simulink library "casper_library_correlator"  (Simulink 8.0)
settings: Solver=ode45  SolverMode=SingleTasking  StartTime=0.0  StopTime=10.0  RelTol=1e-3
values from neighbouring files (symbols this model uses):
  n_bits = eval(get_var('n_bits', 'defaults', defaults, varargin{:}))    [auto_tap_init.m]    (also in baseline_tap_init.m; bi_real_unscr_2x_init.m = get_var('n_bits', 'defaults', defaults, varargin{:}); bi_real_unscr_4x_init.m = get_var('n_bits', 'defaults', defaults, varargin{:}); bit_reverse_init.m = get_var('n_bits',varargin{:}))
libraries: xbsIndex_r4 x1360, casper_library_misc x140, casper_library_multipliers x32, xps_library x8, casper_library_delays x1, casper_library_correlator x1
(part 2 of 14)

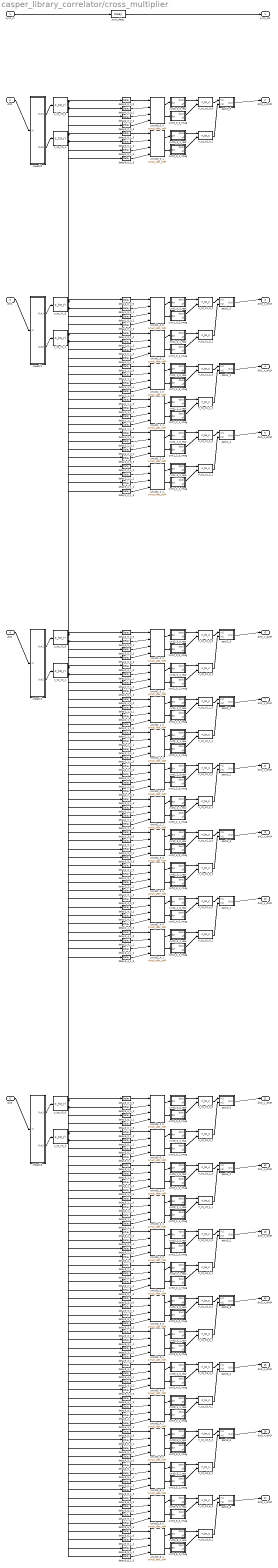
== system casper_library_correlator/cross_multiplier ==
  sync_in : Inport
  din0 : Inport  Port=2
  din1 : Inport  Port=3
  din2 : Inport  Port=4
  din3 : Inport  Port=5
  c_to_ri0_0 : casper_library_misc/c_to_ri  n_bits=bit_width_in  bin_pt=binary_point_in
      settings: AttributesFormatString=4_3 r/i
  c_to_ri0_1 : casper_library_misc/c_to_ri  n_bits=bit_width_in  bin_pt=binary_point_in
      settings: AttributesFormatString=4_3 r/i
  c_to_ri1_0 : casper_library_misc/c_to_ri  n_bits=bit_width_in  bin_pt=binary_point_in
      settings: AttributesFormatString=4_3 r/i
  c_to_ri1_1 : casper_library_misc/c_to_ri  n_bits=bit_width_in  bin_pt=binary_point_in
      settings: AttributesFormatString=4_3 r/i
  c_to_ri2_0 : casper_library_misc/c_to_ri  n_bits=bit_width_in  bin_pt=binary_point_in
      settings: AttributesFormatString=4_3 r/i
  c_to_ri2_1 : casper_library_misc/c_to_ri  n_bits=bit_width_in  bin_pt=binary_point_in
      settings: AttributesFormatString=4_3 r/i
  c_to_ri3_0 : casper_library_misc/c_to_ri  n_bits=bit_width_in  bin_pt=binary_point_in
      settings: AttributesFormatString=4_3 r/i
  c_to_ri3_1 : casper_library_misc/c_to_ri  n_bits=bit_width_in  bin_pt=binary_point_in
      settings: AttributesFormatString=4_3 r/i
  cmult0_0_0 : casper_library_multipliers/cmult_4bit_hdl*  mult_latency=mult_latency  add_latency=add_latency
  cmult0_0_1 : casper_library_multipliers/cmult_4bit_hdl*  mult_latency=mult_latency  add_latency=add_latency
  cmult1_0_0 : casper_library_multipliers/cmult_4bit_hdl*  mult_latency=mult_latency  add_latency=add_latency
  cmult1_0_1 : casper_library_multipliers/cmult_4bit_hdl*  mult_latency=mult_latency  add_latency=add_latency
  cmult1_1_0 : casper_library_multipliers/cmult_4bit_hdl*  mult_latency=mult_latency  add_latency=add_latency
  cmult1_1_1 : casper_library_multipliers/cmult_4bit_hdl*  mult_latency=mult_latency  add_latency=add_latency
  cmult1_2_0 : casper_library_multipliers/cmult_4bit_hdl*  mult_latency=mult_latency  add_latency=add_latency
  cmult1_2_1 : casper_library_multipliers/cmult_4bit_hdl*  mult_latency=mult_latency  add_latency=add_latency
  cmult2_0_0 : casper_library_multipliers/cmult_4bit_hdl*  mult_latency=mult_latency  add_latency=add_latency
  cmult2_0_1 : casper_library_multipliers/cmult_4bit_hdl*  mult_latency=mult_latency  add_latency=add_latency
  cmult2_1_0 : casper_library_multipliers/cmult_4bit_hdl*  mult_latency=mult_latency  add_latency=add_latency
  cmult2_1_1 : casper_library_multipliers/cmult_4bit_hdl*  mult_latency=mult_latency  add_latency=add_latency
  cmult2_2_0 : casper_library_multipliers/cmult_4bit_hdl*  mult_latency=mult_latency  add_latency=add_latency
  cmult2_2_1 : casper_library_multipliers/cmult_4bit_hdl*  mult_latency=mult_latency  add_latency=add_latency
  cmult2_3_0 : casper_library_multipliers/cmult_4bit_hdl*  mult_latency=mult_latency  add_latency=add_latency
  cmult2_3_1 : casper_library_multipliers/cmult_4bit_hdl*  mult_latency=mult_latency  add_latency=add_latency
  cmult2_4_0 : casper_library_multipliers/cmult_4bit_hdl*  mult_latency=mult_latency  add_latency=add_latency
  cmult2_4_1 : casper_library_multipliers/cmult_4bit_hdl*  mult_latency=mult_latency  add_latency=add_latency
  cmult3_0_0 : casper_library_multipliers/cmult_4bit_hdl*  mult_latency=mult_latency  add_latency=add_latency
  cmult3_0_1 : casper_library_multipliers/cmult_4bit_hdl*  mult_latency=mult_latency  add_latency=add_latency
  cmult3_1_0 : casper_library_multipliers/cmult_4bit_hdl*  mult_latency=mult_latency  add_latency=add_latency
  cmult3_1_1 : casper_library_multipliers/cmult_4bit_hdl*  mult_latency=mult_latency  add_latency=add_latency
  cmult3_2_0 : casper_library_multipliers/cmult_4bit_hdl*  mult_latency=mult_latency  add_latency=add_latency
  cmult3_2_1 : casper_library_multipliers/cmult_4bit_hdl*  mult_latency=mult_latency  add_latency=add_latency
  cmult3_3_0 : casper_library_multipliers/cmult_4bit_hdl*  mult_latency=mult_latency  add_latency=add_latency
  cmult3_3_1 : casper_library_multipliers/cmult_4bit_hdl*  mult_latency=mult_latency  add_latency=add_latency
  cmult3_4_0 : casper_library_multipliers/cmult_4bit_hdl*  mult_latency=mult_latency  add_latency=add_latency
  cmult3_4_1 : casper_library_multipliers/cmult_4bit_hdl*  mult_latency=mult_latency  add_latency=add_latency
  cmult3_5_0 : casper_library_multipliers/cmult_4bit_hdl*  mult_latency=mult_latency  add_latency=add_latency
  cmult3_5_1 : casper_library_multipliers/cmult_4bit_hdl*  mult_latency=mult_latency  add_latency=add_latency
  cmult3_6_0 : casper_library_multipliers/cmult_4bit_hdl*  mult_latency=mult_latency  add_latency=add_latency
  cmult3_6_1 : casper_library_multipliers/cmult_4bit_hdl*  mult_latency=mult_latency  add_latency=add_latency
  cvrt0_0_0_imag : Subsystem  AncestorBlock=casper_library_misc/convert_of  mask(convert_of){bit_width_i=9, binary_point_i=6, bit_width_o=9, binary_point_o=6, latency=0, overflow=Wrap, quantization=Truncate}
      mask prompts: bit_width_i "Bit Width In"; binary_point_i "Binary Point In"; bit_width_o "Bit Width Out"; binary_point_o "Binary Point Out"; overflow "Overflow Behaviour"; quantization "Quantization Behaviour"
      mask help:
      | Converts from one 2's complement bit-width
      | and/or binary point position to another.
      | Includes underflow/overflow indicator.
      mask init:
      | convert_of_init(gcb, ...
      |     'bit_width_i', bit_width_i, ...
      |     'binary_point_i', binary_point_i, ...
      |     'bit_width_o', bit_width_o, ...
      |     'binary_point_o', binary_point_o, ...
      |     'latency', latency, ...
      |     'overflow', overflow, ...
      |     'quantization', quantization);
      settings: AttributesFormatString=[9,6]->[9,6]
      mask TypeOptions overflow: Wrap | Saturate | Error
      mask TypeOptions quantization: Truncate | Round  (unbiased: +/- Inf) | Round  (unbiased: even values)
  cvrt0_0_0_real : Subsystem  AncestorBlock=casper_library_misc/convert_of  mask(convert_of){bit_width_i=9, binary_point_i=6, bit_width_o=9, binary_point_o=6, latency=0, overflow=Wrap, quantization=Truncate}
      mask prompts: bit_width_i "Bit Width In"; binary_point_i "Binary Point In"; bit_width_o "Bit Width Out"; binary_point_o "Binary Point Out"; overflow "Overflow Behaviour"; quantization "Quantization Behaviour"
      mask help:
      | Converts from one 2's complement bit-width
      | and/or binary point position to another.
      | Includes underflow/overflow indicator.
      mask init: same as casper_library_correlator/cross_multiplier/cvrt0_0_0_imag
      settings: AttributesFormatString=[9,6]->[9,6]
      mask TypeOptions overflow: Wrap | Saturate | Error
      mask TypeOptions quantization: Truncate | Round  (unbiased: +/- Inf) | Round  (unbiased: even values)
  cvrt0_0_1_imag : Subsystem  AncestorBlock=casper_library_misc/convert_of  mask(convert_of){bit_width_i=9, binary_point_i=6, bit_width_o=9, binary_point_o=6, latency=0, overflow=Wrap, quantization=Truncate}
      mask prompts: bit_width_i "Bit Width In"; binary_point_i "Binary Point In"; bit_width_o "Bit Width Out"; binary_point_o "Binary Point Out"; overflow "Overflow Behaviour"; quantization "Quantization Behaviour"
      mask help:
      | Converts from one 2's complement bit-width
      | and/or binary point position to another.
      | Includes underflow/overflow indicator.
      mask init: same as casper_library_correlator/cross_multiplier/cvrt0_0_0_imag
      settings: AttributesFormatString=[9,6]->[9,6]
      mask TypeOptions overflow: Wrap | Saturate | Error
      mask TypeOptions quantization: Truncate | Round  (unbiased: +/- Inf) | Round  (unbiased: even values)
  cvrt0_0_1_real : Subsystem  AncestorBlock=casper_library_misc/convert_of  mask(convert_of){bit_width_i=9, binary_point_i=6, bit_width_o=9, binary_point_o=6, latency=0, overflow=Wrap, quantization=Truncate}
      mask prompts: bit_width_i "Bit Width In"; binary_point_i "Binary Point In"; bit_width_o "Bit Width Out"; binary_point_o "Binary Point Out"; overflow "Overflow Behaviour"; quantization "Quantization Behaviour"
      mask help:
      | Converts from one 2's complement bit-width
      | and/or binary point position to another.
      | Includes underflow/overflow indicator.
      mask init: same as casper_library_correlator/cross_multiplier/cvrt0_0_0_imag
      settings: AttributesFormatString=[9,6]->[9,6]
      mask TypeOptions overflow: Wrap | Saturate | Error
      mask TypeOptions quantization: Truncate | Round  (unbiased: +/- Inf) | Round  (unbiased: even values)
  cvrt1_0_0_imag : Subsystem  AncestorBlock=casper_library_misc/convert_of  mask(convert_of){bit_width_i=9, binary_point_i=6, bit_width_o=9, binary_point_o=6, latency=0, overflow=Wrap, quantization=Truncate}
      mask prompts: bit_width_i "Bit Width In"; binary_point_i "Binary Point In"; bit_width_o "Bit Width Out"; binary_point_o "Binary Point Out"; overflow "Overflow Behaviour"; quantization "Quantization Behaviour"
      mask help:
      | Converts from one 2's complement bit-width
      | and/or binary point position to another.
      | Includes underflow/overflow indicator.
      mask init: same as casper_library_correlator/cross_multiplier/cvrt0_0_0_imag
      settings: AttributesFormatString=[9,6]->[9,6]
      mask TypeOptions overflow: Wrap | Saturate | Error
      mask TypeOptions quantization: Truncate | Round  (unbiased: +/- Inf) | Round  (unbiased: even values)
  cvrt1_0_0_real : Subsystem  AncestorBlock=casper_library_misc/convert_of  mask(convert_of){bit_width_i=9, binary_point_i=6, bit_width_o=9, binary_point_o=6, latency=0, overflow=Wrap, quantization=Truncate}
      mask prompts: bit_width_i "Bit Width In"; binary_point_i "Binary Point In"; bit_width_o "Bit Width Out"; binary_point_o "Binary Point Out"; overflow "Overflow Behaviour"; quantization "Quantization Behaviour"
      mask help:
      | Converts from one 2's complement bit-width
      | and/or binary point position to another.
      | Includes underflow/overflow indicator.
      mask init: same as casper_library_correlator/cross_multiplier/cvrt0_0_0_imag
      settings: AttributesFormatString=[9,6]->[9,6]
      mask TypeOptions overflow: Wrap | Saturate | Error
      mask TypeOptions quantization: Truncate | Round  (unbiased: +/- Inf) | Round  (unbiased: even values)
  cvrt1_0_1_imag : Subsystem  AncestorBlock=casper_library_misc/convert_of  mask(convert_of){bit_width_i=9, binary_point_i=6, bit_width_o=9, binary_point_o=6, latency=0, overflow=Wrap, quantization=Truncate}
      mask prompts: bit_width_i "Bit Width In"; binary_point_i "Binary Point In"; bit_width_o "Bit Width Out"; binary_point_o "Binary Point Out"; overflow "Overflow Behaviour"; quantization "Quantization Behaviour"
      mask help:
      | Converts from one 2's complement bit-width
      | and/or binary point position to another.
      | Includes underflow/overflow indicator.
      mask init: same as casper_library_correlator/cross_multiplier/cvrt0_0_0_imag
      settings: AttributesFormatString=[9,6]->[9,6]
      mask TypeOptions overflow: Wrap | Saturate | Error
      mask TypeOptions quantization: Truncate | Round  (unbiased: +/- Inf) | Round  (unbiased: even values)
  cvrt1_0_1_real : Subsystem  AncestorBlock=casper_library_misc/convert_of  mask(convert_of){bit_width_i=9, binary_point_i=6, bit_width_o=9, binary_point_o=6, latency=0, overflow=Wrap, quantization=Truncate}
      mask prompts: bit_width_i "Bit Width In"; binary_point_i "Binary Point In"; bit_width_o "Bit Width Out"; binary_point_o "Binary Point Out"; overflow "Overflow Behaviour"; quantization "Quantization Behaviour"
      mask help:
      | Converts from one 2's complement bit-width
      | and/or binary point position to another.
      | Includes underflow/overflow indicator.
      mask init: same as casper_library_correlator/cross_multiplier/cvrt0_0_0_imag
      settings: AttributesFormatString=[9,6]->[9,6]
      mask TypeOptions overflow: Wrap | Saturate | Error
      mask TypeOptions quantization: Truncate | Round  (unbiased: +/- Inf) | Round  (unbiased: even values)
  cvrt1_1_0_imag : Subsystem  AncestorBlock=casper_library_misc/convert_of  mask(convert_of){bit_width_i=9, binary_point_i=6, bit_width_o=9, binary_point_o=6, latency=0, overflow=Wrap, quantization=Truncate}
      mask prompts: bit_width_i "Bit Width In"; binary_point_i "Binary Point In"; bit_width_o "Bit Width Out"; binary_point_o "Binary Point Out"; overflow "Overflow Behaviour"; quantization "Quantization Behaviour"
      mask help:
      | Converts from one 2's complement bit-width
      | and/or binary point position to another.
      | Includes underflow/overflow indicator.
      mask init: same as casper_library_correlator/cross_multiplier/cvrt0_0_0_imag
      settings: AttributesFormatString=[9,6]->[9,6]
      mask TypeOptions overflow: Wrap | Saturate | Error
      mask TypeOptions quantization: Truncate | Round  (unbiased: +/- Inf) | Round  (unbiased: even values)
  cvrt1_1_0_real : Subsystem  AncestorBlock=casper_library_misc/convert_of  mask(convert_of){bit_width_i=9, binary_point_i=6, bit_width_o=9, binary_point_o=6, latency=0, overflow=Wrap, quantization=Truncate}
      mask prompts: bit_width_i "Bit Width In"; binary_point_i "Binary Point In"; bit_width_o "Bit Width Out"; binary_point_o "Binary Point Out"; overflow "Overflow Behaviour"; quantization "Quantization Behaviour"
      mask help:
      | Converts from one 2's complement bit-width
      | and/or binary point position to another.
      | Includes underflow/overflow indicator.
      mask init: same as casper_library_correlator/cross_multiplier/cvrt0_0_0_imag
      settings: AttributesFormatString=[9,6]->[9,6]
      mask TypeOptions overflow: Wrap | Saturate | Error
      mask TypeOptions quantization: Truncate | Round  (unbiased: +/- Inf) | Round  (unbiased: even values)
  cvrt1_1_1_imag : Subsystem  AncestorBlock=casper_library_misc/convert_of  mask(convert_of){bit_width_i=9, binary_point_i=6, bit_width_o=9, binary_point_o=6, latency=0, overflow=Wrap, quantization=Truncate}
      mask prompts: bit_width_i "Bit Width In"; binary_point_i "Binary Point In"; bit_width_o "Bit Width Out"; binary_point_o "Binary Point Out"; overflow "Overflow Behaviour"; quantization "Quantization Behaviour"
      mask help:
      | Converts from one 2's complement bit-width
      | and/or binary point position to another.
      | Includes underflow/overflow indicator.
      mask init: same as casper_library_correlator/cross_multiplier/cvrt0_0_0_imag
      settings: AttributesFormatString=[9,6]->[9,6]
      mask TypeOptions overflow: Wrap | Saturate | Error
      mask TypeOptions quantization: Truncate | Round  (unbiased: +/- Inf) | Round  (unbiased: even values)
  cvrt1_1_1_real : Subsystem  AncestorBlock=casper_library_misc/convert_of  mask(convert_of){bit_width_i=9, binary_point_i=6, bit_width_o=9, binary_point_o=6, latency=0, overflow=Wrap, quantization=Truncate}
      mask prompts: bit_width_i "Bit Width In"; binary_point_i "Binary Point In"; bit_width_o "Bit Width Out"; binary_point_o "Binary Point Out"; overflow "Overflow Behaviour"; quantization "Quantization Behaviour"
      mask help:
      | Converts from one 2's complement bit-width
      | and/or binary point position to another.
      | Includes underflow/overflow indicator.
      mask init: same as casper_library_correlator/cross_multiplier/cvrt0_0_0_imag
      settings: AttributesFormatString=[9,6]->[9,6]
      mask TypeOptions overflow: Wrap | Saturate | Error
      mask TypeOptions quantization: Truncate | Round  (unbiased: +/- Inf) | Round  (unbiased: even values)
  cvrt1_2_0_imag : Subsystem  AncestorBlock=casper_library_misc/convert_of  mask(convert_of){bit_width_i=9, binary_point_i=6, bit_width_o=9, binary_point_o=6, latency=0, overflow=Wrap, quantization=Truncate}
      mask prompts: bit_width_i "Bit Width In"; binary_point_i "Binary Point In"; bit_width_o "Bit Width Out"; binary_point_o "Binary Point Out"; overflow "Overflow Behaviour"; quantization "Quantization Behaviour"
      mask help:
      | Converts from one 2's complement bit-width
      | and/or binary point position to another.
      | Includes underflow/overflow indicator.
      mask init: same as casper_library_correlator/cross_multiplier/cvrt0_0_0_imag
      settings: AttributesFormatString=[9,6]->[9,6]
      mask TypeOptions overflow: Wrap | Saturate | Error
      mask TypeOptions quantization: Truncate | Round  (unbiased: +/- Inf) | Round  (unbiased: even values)
  cvrt1_2_0_real : Subsystem  AncestorBlock=casper_library_misc/convert_of  mask(convert_of){bit_width_i=9, binary_point_i=6, bit_width_o=9, binary_point_o=6, latency=0, overflow=Wrap, quantization=Truncate}
      mask prompts: bit_width_i "Bit Width In"; binary_point_i "Binary Point In"; bit_width_o "Bit Width Out"; binary_point_o "Binary Point Out"; overflow "Overflow Behaviour"; quantization "Quantization Behaviour"
      mask help:
      | Converts from one 2's complement bit-width
      | and/or binary point position to another.
      | Includes underflow/overflow indicator.
      mask init: same as casper_library_correlator/cross_multiplier/cvrt0_0_0_imag
      settings: AttributesFormatString=[9,6]->[9,6]
      mask TypeOptions overflow: Wrap | Saturate | Error
      mask TypeOptions quantization: Truncate | Round  (unbiased: +/- Inf) | Round  (unbiased: even values)
  cvrt1_2_1_imag : Subsystem  AncestorBlock=casper_library_misc/convert_of  mask(convert_of){bit_width_i=9, binary_point_i=6, bit_width_o=9, binary_point_o=6, latency=0, overflow=Wrap, quantization=Truncate}
      mask prompts: bit_width_i "Bit Width In"; binary_point_i "Binary Point In"; bit_width_o "Bit Width Out"; binary_point_o "Binary Point Out"; overflow "Overflow Behaviour"; quantization "Quantization Behaviour"
      mask help:
      | Converts from one 2's complement bit-width
      | and/or binary point position to another.
      | Includes underflow/overflow indicator.
      mask init: same as casper_library_correlator/cross_multiplier/cvrt0_0_0_imag
      settings: AttributesFormatString=[9,6]->[9,6]
      mask TypeOptions overflow: Wrap | Saturate | Error
      mask TypeOptions quantization: Truncate | Round  (unbiased: +/- Inf) | Round  (unbiased: even values)
  cvrt1_2_1_real : Subsystem  AncestorBlock=casper_library_misc/convert_of  mask(convert_of){bit_width_i=9, binary_point_i=6, bit_width_o=9, binary_point_o=6, latency=0, overflow=Wrap, quantization=Truncate}
      mask prompts: bit_width_i "Bit Width In"; binary_point_i "Binary Point In"; bit_width_o "Bit Width Out"; binary_point_o "Binary Point Out"; overflow "Overflow Behaviour"; quantization "Quantization Behaviour"
      mask help:
      | Converts from one 2's complement bit-width
      | and/or binary point position to another.
      | Includes underflow/overflow indicator.
      mask init: same as casper_library_correlator/cross_multiplier/cvrt0_0_0_imag
      settings: AttributesFormatString=[9,6]->[9,6]
      mask TypeOptions overflow: Wrap | Saturate | Error
      mask TypeOptions quantization: Truncate | Round  (unbiased: +/- Inf) | Round  (unbiased: even values)
  cvrt2_0_0_imag : Subsystem  AncestorBlock=casper_library_misc/convert_of  mask(convert_of){bit_width_i=9, binary_point_i=6, bit_width_o=9, binary_point_o=6, latency=0, overflow=Wrap, quantization=Truncate}
      mask prompts: bit_width_i "Bit Width In"; binary_point_i "Binary Point In"; bit_width_o "Bit Width Out"; binary_point_o "Binary Point Out"; overflow "Overflow Behaviour"; quantization "Quantization Behaviour"
      mask help:
      | Converts from one 2's complement bit-width
      | and/or binary point position to another.
      | Includes underflow/overflow indicator.
      mask init: same as casper_library_correlator/cross_multiplier/cvrt0_0_0_imag
      settings: AttributesFormatString=[9,6]->[9,6]
      mask TypeOptions overflow: Wrap | Saturate | Error
      mask TypeOptions quantization: Truncate | Round  (unbiased: +/- Inf) | Round  (unbiased: even values)
  cvrt2_0_0_real : Subsystem  AncestorBlock=casper_library_misc/convert_of  mask(convert_of){bit_width_i=9, binary_point_i=6, bit_width_o=9, binary_point_o=6, latency=0, overflow=Wrap, quantization=Truncate}
      mask prompts: bit_width_i "Bit Width In"; binary_point_i "Binary Point In"; bit_width_o "Bit Width Out"; binary_point_o "Binary Point Out"; overflow "Overflow Behaviour"; quantization "Quantization Behaviour"
      mask help:
      | Converts from one 2's complement bit-width
      | and/or binary point position to another.
      | Includes underflow/overflow indicator.
      mask init: same as casper_library_correlator/cross_multiplier/cvrt0_0_0_imag
      settings: AttributesFormatString=[9,6]->[9,6]
      mask TypeOptions overflow: Wrap | Saturate | Error
      mask TypeOptions quantization: Truncate | Round  (unbiased: +/- Inf) | Round  (unbiased: even values)
  cvrt2_0_1_imag : Subsystem  AncestorBlock=casper_library_misc/convert_of  mask(convert_of){bit_width_i=9, binary_point_i=6, bit_width_o=9, binary_point_o=6, latency=0, overflow=Wrap, quantization=Truncate}
      mask prompts: bit_width_i "Bit Width In"; binary_point_i "Binary Point In"; bit_width_o "Bit Width Out"; binary_point_o "Binary Point Out"; overflow "Overflow Behaviour"; quantization "Quantization Behaviour"
      mask help:
      | Converts from one 2's complement bit-width
      | and/or binary point position to another.
      | Includes underflow/overflow indicator.
      mask init: same as casper_library_correlator/cross_multiplier/cvrt0_0_0_imag
      settings: AttributesFormatString=[9,6]->[9,6]
      mask TypeOptions overflow: Wrap | Saturate | Error
      mask TypeOptions quantization: Truncate | Round  (unbiased: +/- Inf) | Round  (unbiased: even values)
  cvrt2_0_1_real : Subsystem  AncestorBlock=casper_library_misc/convert_of  mask(convert_of){bit_width_i=9, binary_point_i=6, bit_width_o=9, binary_point_o=6, latency=0, overflow=Wrap, quantization=Truncate}
      mask prompts: bit_width_i "Bit Width In"; binary_point_i "Binary Point In"; bit_width_o "Bit Width Out"; binary_point_o "Binary Point Out"; overflow "Overflow Behaviour"; quantization "Quantization Behaviour"
      mask help:
      | Converts from one 2's complement bit-width
      | and/or binary point position to another.
      | Includes underflow/overflow indicator.
      mask init: same as casper_library_correlator/cross_multiplier/cvrt0_0_0_imag
      settings: AttributesFormatString=[9,6]->[9,6]
      mask TypeOptions overflow: Wrap | Saturate | Error
      mask TypeOptions quantization: Truncate | Round  (unbiased: +/- Inf) | Round  (unbiased: even values)
  cvrt2_1_0_imag : Subsystem  AncestorBlock=casper_library_misc/convert_of  mask(convert_of){bit_width_i=9, binary_point_i=6, bit_width_o=9, binary_point_o=6, latency=0, overflow=Wrap, quantization=Truncate}
      mask prompts: bit_width_i "Bit Width In"; binary_point_i "Binary Point In"; bit_width_o "Bit Width Out"; binary_point_o "Binary Point Out"; overflow "Overflow Behaviour"; quantization "Quantization Behaviour"
      mask help:
      | Converts from one 2's complement bit-width
      | and/or binary point position to another.
      | Includes underflow/overflow indicator.
      mask init: same as casper_library_correlator/cross_multiplier/cvrt0_0_0_imag
      settings: AttributesFormatString=[9,6]->[9,6]
      mask TypeOptions overflow: Wrap | Saturate | Error
      mask TypeOptions quantization: Truncate | Round  (unbiased: +/- Inf) | Round  (unbiased: even values)
  cvrt2_1_0_real : Subsystem  AncestorBlock=casper_library_misc/convert_of  mask(convert_of){bit_width_i=9, binary_point_i=6, bit_width_o=9, binary_point_o=6, latency=0, overflow=Wrap, quantization=Truncate}
      mask prompts: bit_width_i "Bit Width In"; binary_point_i "Binary Point In"; bit_width_o "Bit Width Out"; binary_point_o "Binary Point Out"; overflow "Overflow Behaviour"; quantization "Quantization Behaviour"
      mask help:
      | Converts from one 2's complement bit-width
      | and/or binary point position to another.
      | Includes underflow/overflow indicator.
      mask init: same as casper_library_correlator/cross_multiplier/cvrt0_0_0_imag
      settings: AttributesFormatString=[9,6]->[9,6]
      mask TypeOptions overflow: Wrap | Saturate | Error
      mask TypeOptions quantization: Truncate | Round  (unbiased: +/- Inf) | Round  (unbiased: even values)
  cvrt2_1_1_imag : Subsystem  AncestorBlock=casper_library_misc/convert_of  mask(convert_of){bit_width_i=9, binary_point_i=6, bit_width_o=9, binary_point_o=6, latency=0, overflow=Wrap, quantization=Truncate}
      mask prompts: bit_width_i "Bit Width In"; binary_point_i "Binary Point In"; bit_width_o "Bit Width Out"; binary_point_o "Binary Point Out"; overflow "Overflow Behaviour"; quantization "Quantization Behaviour"
      mask help:
      | Converts from one 2's complement bit-width
      | and/or binary point position to another.
      | Includes underflow/overflow indicator.
      mask init: same as casper_library_correlator/cross_multiplier/cvrt0_0_0_imag
      settings: AttributesFormatString=[9,6]->[9,6]
      mask TypeOptions overflow: Wrap | Saturate | Error
      mask TypeOptions quantization: Truncate | Round  (unbiased: +/- Inf) | Round  (unbiased: even values)
  cvrt2_1_1_real : Subsystem  AncestorBlock=casper_library_misc/convert_of  mask(convert_of){bit_width_i=9, binary_point_i=6, bit_width_o=9, binary_point_o=6, latency=0, overflow=Wrap, quantization=Truncate}
      mask prompts: bit_width_i "Bit Width In"; binary_point_i "Binary Point In"; bit_width_o "Bit Width Out"; binary_point_o "Binary Point Out"; overflow "Overflow Behaviour"; quantization "Quantization Behaviour"
      mask help:
      | Converts from one 2's complement bit-width
      | and/or binary point position to another.
      | Includes underflow/overflow indicator.
      mask init: same as casper_library_correlator/cross_multiplier/cvrt0_0_0_imag
      settings: AttributesFormatString=[9,6]->[9,6]
      mask TypeOptions overflow: Wrap | Saturate | Error
      mask TypeOptions quantization: Truncate | Round  (unbiased: +/- Inf) | Round  (unbiased: even values)
  cvrt2_2_0_imag : Subsystem  AncestorBlock=casper_library_misc/convert_of  mask(convert_of){bit_width_i=9, binary_point_i=6, bit_width_o=9, binary_point_o=6, latency=0, overflow=Wrap, quantization=Truncate}
      mask prompts: bit_width_i "Bit Width In"; binary_point_i "Binary Point In"; bit_width_o "Bit Width Out"; binary_point_o "Binary Point Out"; overflow "Overflow Behaviour"; quantization "Quantization Behaviour"
      mask help:
      | Converts from one 2's complement bit-width
      | and/or binary point position to another.
      | Includes underflow/overflow indicator.
      mask init: same as casper_library_correlator/cross_multiplier/cvrt0_0_0_imag
      settings: AttributesFormatString=[9,6]->[9,6]
      mask TypeOptions overflow: Wrap | Saturate | Error
      mask TypeOptions quantization: Truncate | Round  (unbiased: +/- Inf) | Round  (unbiased: even values)
  cvrt2_2_0_real : Subsystem  AncestorBlock=casper_library_misc/convert_of  mask(convert_of){bit_width_i=9, binary_point_i=6, bit_width_o=9, binary_point_o=6, latency=0, overflow=Wrap, quantization=Truncate}
      mask prompts: bit_width_i "Bit Width In"; binary_point_i "Binary Point In"; bit_width_o "Bit Width Out"; binary_point_o "Binary Point Out"; overflow "Overflow Behaviour"; quantization "Quantization Behaviour"
      mask help:
      | Converts from one 2's complement bit-width
      | and/or binary point position to another.
      | Includes underflow/overflow indicator.
      mask init: same as casper_library_correlator/cross_multiplier/cvrt0_0_0_imag
      settings: AttributesFormatString=[9,6]->[9,6]
      mask TypeOptions overflow: Wrap | Saturate | Error
      mask TypeOptions quantization: Truncate | Round  (unbiased: +/- Inf) | Round  (unbiased: even values)
  cvrt2_2_1_imag : Subsystem  AncestorBlock=casper_library_misc/convert_of  mask(convert_of){bit_width_i=9, binary_point_i=6, bit_width_o=9, binary_point_o=6, latency=0, overflow=Wrap, quantization=Truncate}
      mask prompts: bit_width_i "Bit Width In"; binary_point_i "Binary Point In"; bit_width_o "Bit Width Out"; binary_point_o "Binary Point Out"; overflow "Overflow Behaviour"; quantization "Quantization Behaviour"
      mask help:
      | Converts from one 2's complement bit-width
      | and/or binary point position to another.
      | Includes underflow/overflow indicator.
      mask init: same as casper_library_correlator/cross_multiplier/cvrt0_0_0_imag
      settings: AttributesFormatString=[9,6]->[9,6]
      mask TypeOptions overflow: Wrap | Saturate | Error
      mask TypeOptions quantization: Truncate | Round  (unbiased: +/- Inf) | Round  (unbiased: even values)
  cvrt2_2_1_real : Subsystem  AncestorBlock=casper_library_misc/convert_of  mask(convert_of){bit_width_i=9, binary_point_i=6, bit_width_o=9, binary_point_o=6, latency=0, overflow=Wrap, quantization=Truncate}
      mask prompts: bit_width_i "Bit Width In"; binary_point_i "Binary Point In"; bit_width_o "Bit Width Out"; binary_point_o "Binary Point Out"; overflow "Overflow Behaviour"; quantization "Quantization Behaviour"
      mask help:
      | Converts from one 2's complement bit-width
      | and/or binary point position to another.
      | Includes underflow/overflow indicator.
      mask init: same as casper_library_correlator/cross_multiplier/cvrt0_0_0_imag
      settings: AttributesFormatString=[9,6]->[9,6]
      mask TypeOptions overflow: Wrap | Saturate | Error
      mask TypeOptions quantization: Truncate | Round  (unbiased: +/- Inf) | Round  (unbiased: even values)
  cvrt2_3_0_imag : Subsystem  AncestorBlock=casper_library_misc/convert_of  mask(convert_of){bit_width_i=9, binary_point_i=6, bit_width_o=9, binary_point_o=6, latency=0, overflow=Wrap, quantization=Truncate}
      mask prompts: bit_width_i "Bit Width In"; binary_point_i "Binary Point In"; bit_width_o "Bit Width Out"; binary_point_o "Binary Point Out"; overflow "Overflow Behaviour"; quantization "Quantization Behaviour"
      mask help:
      | Converts from one 2's complement bit-width
      | and/or binary point position to another.
      | Includes underflow/overflow indicator.
      mask init: same as casper_library_correlator/cross_multiplier/cvrt0_0_0_imag
      settings: AttributesFormatString=[9,6]->[9,6]
      mask TypeOptions overflow: Wrap | Saturate | Error
      mask TypeOptions quantization: Truncate | Round  (unbiased: +/- Inf) | Round  (unbiased: even values)
  cvrt2_3_0_real : Subsystem  AncestorBlock=casper_library_misc/convert_of  mask(convert_of){bit_width_i=9, binary_point_i=6, bit_width_o=9, binary_point_o=6, latency=0, overflow=Wrap, quantization=Truncate}
      mask prompts: bit_width_i "Bit Width In"; binary_point_i "Binary Point In"; bit_width_o "Bit Width Out"; binary_point_o "Binary Point Out"; overflow "Overflow Behaviour"; quantization "Quantization Behaviour"
      mask help:
      | Converts from one 2's complement bit-width
      | and/or binary point position to another.
      | Includes underflow/overflow indicator.
      mask init: same as casper_library_correlator/cross_multiplier/cvrt0_0_0_imag
      settings: AttributesFormatString=[9,6]->[9,6]
      mask TypeOptions overflow: Wrap | Saturate | Error
      mask TypeOptions quantization: Truncate | Round  (unbiased: +/- Inf) | Round  (unbiased: even values)
  cvrt2_3_1_imag : Subsystem  AncestorBlock=casper_library_misc/convert_of  mask(convert_of){bit_width_i=9, binary_point_i=6, bit_width_o=9, binary_point_o=6, latency=0, overflow=Wrap, quantization=Truncate}
      mask prompts: bit_width_i "Bit Width In"; binary_point_i "Binary Point In"; bit_width_o "Bit Width Out"; binary_point_o "Binary Point Out"; overflow "Overflow Behaviour"; quantization "Quantization Behaviour"
      mask help:
      | Converts from one 2's complement bit-width
      | and/or binary point position to another.
      | Includes underflow/overflow indicator.
      mask init: same as casper_library_correlator/cross_multiplier/cvrt0_0_0_imag
      settings: AttributesFormatString=[9,6]->[9,6]
      mask TypeOptions overflow: Wrap | Saturate | Error
      mask TypeOptions quantization: Truncate | Round  (unbiased: +/- Inf) | Round  (unbiased: even values)
  cvrt2_3_1_real : Subsystem  AncestorBlock=casper_library_misc/convert_of  mask(convert_of){bit_width_i=9, binary_point_i=6, bit_width_o=9, binary_point_o=6, latency=0, overflow=Wrap, quantization=Truncate}
      mask prompts: bit_width_i "Bit Width In"; binary_point_i "Binary Point In"; bit_width_o "Bit Width Out"; binary_point_o "Binary Point Out"; overflow "Overflow Behaviour"; quantization "Quantization Behaviour"
      mask help:
      | Converts from one 2's complement bit-width
      | and/or binary point position to another.
      | Includes underflow/overflow indicator.
      mask init: same as casper_library_correlator/cross_multiplier/cvrt0_0_0_imag
      settings: AttributesFormatString=[9,6]->[9,6]
      mask TypeOptions overflow: Wrap | Saturate | Error
      mask TypeOptions quantization: Truncate | Round  (unbiased: +/- Inf) | Round  (unbiased: even values)
  cvrt2_4_0_imag : Subsystem  AncestorBlock=casper_library_misc/convert_of  mask(convert_of){bit_width_i=9, binary_point_i=6, bit_width_o=9, binary_point_o=6, latency=0, overflow=Wrap, quantization=Truncate}
      mask prompts: bit_width_i "Bit Width In"; binary_point_i "Binary Point In"; bit_width_o "Bit Width Out"; binary_point_o "Binary Point Out"; overflow "Overflow Behaviour"; quantization "Quantization Behaviour"
      mask help:
      | Converts from one 2's complement bit-width
      | and/or binary point position to another.
      | Includes underflow/overflow indicator.
      mask init: same as casper_library_correlator/cross_multiplier/cvrt0_0_0_imag
      settings: AttributesFormatString=[9,6]->[9,6]
      mask TypeOptions overflow: Wrap | Saturate | Error
      mask TypeOptions quantization: Truncate | Round  (unbiased: +/- Inf) | Round  (unbiased: even values)
  cvrt2_4_0_real : Subsystem  AncestorBlock=casper_library_misc/convert_of  mask(convert_of){bit_width_i=9, binary_point_i=6, bit_width_o=9, binary_point_o=6, latency=0, overflow=Wrap, quantization=Truncate}
      mask prompts: bit_width_i "Bit Width In"; binary_point_i "Binary Point In"; bit_width_o "Bit Width Out"; binary_point_o "Binary Point Out"; overflow "Overflow Behaviour"; quantization "Quantization Behaviour"
      mask help:
      | Converts from one 2's complement bit-width
      | and/or binary point position to another.
      | Includes underflow/overflow indicator.
      mask init: same as casper_library_correlator/cross_multiplier/cvrt0_0_0_imag
      settings: AttributesFormatString=[9,6]->[9,6]
      mask TypeOptions overflow: Wrap | Saturate | Error
      mask TypeOptions quantization: Truncate | Round  (unbiased: +/- Inf) | Round  (unbiased: even values)
  cvrt2_4_1_imag : Subsystem  AncestorBlock=casper_library_misc/convert_of  mask(convert_of){bit_width_i=9, binary_point_i=6, bit_width_o=9, binary_point_o=6, latency=0, overflow=Wrap, quantization=Truncate}
      mask prompts: bit_width_i "Bit Width In"; binary_point_i "Binary Point In"; bit_width_o "Bit Width Out"; binary_point_o "Binary Point Out"; overflow "Overflow Behaviour"; quantization "Quantization Behaviour"
      mask help:
      | Converts from one 2's complement bit-width
      | and/or binary point position to another.
      | Includes underflow/overflow indicator.
      mask init: same as casper_library_correlator/cross_multiplier/cvrt0_0_0_imag
      settings: AttributesFormatString=[9,6]->[9,6]
      mask TypeOptions overflow: Wrap | Saturate | Error
      mask TypeOptions quantization: Truncate | Round  (unbiased: +/- Inf) | Round  (unbiased: even values)
  cvrt2_4_1_real : Subsystem  AncestorBlock=casper_library_misc/convert_of  mask(convert_of){bit_width_i=9, binary_point_i=6, bit_width_o=9, binary_point_o=6, latency=0, overflow=Wrap, quantization=Truncate}
      mask prompts: bit_width_i "Bit Width In"; binary_point_i "Binary Point In"; bit_width_o "Bit Width Out"; binary_point_o "Binary Point Out"; overflow "Overflow Behaviour"; quantization "Quantization Behaviour"
      mask help:
      | Converts from one 2's complement bit-width
      | and/or binary point position to another.
      | Includes underflow/overflow indicator.
      mask init: same as casper_library_correlator/cross_multiplier/cvrt0_0_0_imag
      settings: AttributesFormatString=[9,6]->[9,6]
      mask TypeOptions overflow: Wrap | Saturate | Error
      mask TypeOptions quantization: Truncate | Round  (unbiased: +/- Inf) | Round  (unbiased: even values)
  cvrt3_0_0_imag : Subsystem  AncestorBlock=casper_library_misc/convert_of  mask(convert_of){bit_width_i=9, binary_point_i=6, bit_width_o=9, binary_point_o=6, latency=0, overflow=Wrap, quantization=Truncate}
      mask prompts: bit_width_i "Bit Width In"; binary_point_i "Binary Point In"; bit_width_o "Bit Width Out"; binary_point_o "Binary Point Out"; overflow "Overflow Behaviour"; quantization "Quantization Behaviour"
      mask help:
      | Converts from one 2's complement bit-width
      | and/or binary point position to another.
      | Includes underflow/overflow indicator.
      mask init: same as casper_library_correlator/cross_multiplier/cvrt0_0_0_imag
      settings: AttributesFormatString=[9,6]->[9,6]
      mask TypeOptions overflow: Wrap | Saturate | Error
      mask TypeOptions quantization: Truncate | Round  (unbiased: +/- Inf) | Round  (unbiased: even values)
  cvrt3_0_0_real : Subsystem  AncestorBlock=casper_library_misc/convert_of  mask(convert_of){bit_width_i=9, binary_point_i=6, bit_width_o=9, binary_point_o=6, latency=0, overflow=Wrap, quantization=Truncate}
      mask prompts: bit_width_i "Bit Width In"; binary_point_i "Binary Point In"; bit_width_o "Bit Width Out"; binary_point_o "Binary Point Out"; overflow "Overflow Behaviour"; quantization "Quantization Behaviour"
      mask help:
      | Converts from one 2's complement bit-width
      | and/or binary point position to another.
      | Includes underflow/overflow indicator.
      mask init: same as casper_library_correlator/cross_multiplier/cvrt0_0_0_imag
      settings: AttributesFormatString=[9,6]->[9,6]
      mask TypeOptions overflow: Wrap | Saturate | Error
      mask TypeOptions quantization: Truncate | Round  (unbiased: +/- Inf) | Round  (unbiased: even values)
  cvrt3_0_1_imag : Subsystem  AncestorBlock=casper_library_misc/convert_of  mask(convert_of){bit_width_i=9, binary_point_i=6, bit_width_o=9, binary_point_o=6, latency=0, overflow=Wrap, quantization=Truncate}
      mask prompts: bit_width_i "Bit Width In"; binary_point_i "Binary Point In"; bit_width_o "Bit Width Out"; binary_point_o "Binary Point Out"; overflow "Overflow Behaviour"; quantization "Quantization Behaviour"
      mask help:
      | Converts from one 2's complement bit-width
      | and/or binary point position to another.
      | Includes underflow/overflow indicator.
      mask init: same as casper_library_correlator/cross_multiplier/cvrt0_0_0_imag
      settings: AttributesFormatString=[9,6]->[9,6]
      mask TypeOptions overflow: Wrap | Saturate | Error
      mask TypeOptions quantization: Truncate | Round  (unbiased: +/- Inf) | Round  (unbiased: even values)
  cvrt3_0_1_real : Subsystem  AncestorBlock=casper_library_misc/convert_of  mask(convert_of){bit_width_i=9, binary_point_i=6, bit_width_o=9, binary_point_o=6, latency=0, overflow=Wrap, quantization=Truncate}
      mask prompts: bit_width_i "Bit Width In"; binary_point_i "Binary Point In"; bit_width_o "Bit Width Out"; binary_point_o "Binary Point Out"; overflow "Overflow Behaviour"; quantization "Quantization Behaviour"
      mask help:
      | Converts from one 2's complement bit-width
      | and/or binary point position to another.
      | Includes underflow/overflow indicator.
      mask init: same as casper_library_correlator/cross_multiplier/cvrt0_0_0_imag
      settings: AttributesFormatString=[9,6]->[9,6]
      mask TypeOptions overflow: Wrap | Saturate | Error
      mask TypeOptions quantization: Truncate | Round  (unbiased: +/- Inf) | Round  (unbiased: even values)
  cvrt3_1_0_imag : Subsystem  AncestorBlock=casper_library_misc/convert_of  mask(convert_of){bit_width_i=9, binary_point_i=6, bit_width_o=9, binary_point_o=6, latency=0, overflow=Wrap, quantization=Truncate}
      mask prompts: bit_width_i "Bit Width In"; binary_point_i "Binary Point In"; bit_width_o "Bit Width Out"; binary_point_o "Binary Point Out"; overflow "Overflow Behaviour"; quantization "Quantization Behaviour"
      mask help:
      | Converts from one 2's complement bit-width
      | and/or binary point position to another.
      | Includes underflow/overflow indicator.
      mask init: same as casper_library_correlator/cross_multiplier/cvrt0_0_0_imag
      settings: AttributesFormatString=[9,6]->[9,6]
      mask TypeOptions overflow: Wrap | Saturate | Error
      mask TypeOptions quantization: Truncate | Round  (unbiased: +/- Inf) | Round  (unbiased: even values)
  cvrt3_1_0_real : Subsystem  AncestorBlock=casper_library_misc/convert_of  mask(convert_of){bit_width_i=9, binary_point_i=6, bit_width_o=9, binary_point_o=6, latency=0, overflow=Wrap, quantization=Truncate}
      mask prompts: bit_width_i "Bit Width In"; binary_point_i "Binary Point In"; bit_width_o "Bit Width Out"; binary_point_o "Binary Point Out"; overflow "Overflow Behaviour"; quantization "Quantization Behaviour"
      mask help:
      | Converts from one 2's complement bit-width
      | and/or binary point position to another.
      | Includes underflow/overflow indicator.
      mask init: same as casper_library_correlator/cross_multiplier/cvrt0_0_0_imag
      settings: AttributesFormatString=[9,6]->[9,6]
      mask TypeOptions overflow: Wrap | Saturate | Error
      mask TypeOptions quantization: Truncate | Round  (unbiased: +/- Inf) | Round  (unbiased: even values)
  cvrt3_1_1_imag : Subsystem  AncestorBlock=casper_library_misc/convert_of  mask(convert_of){bit_width_i=9, binary_point_i=6, bit_width_o=9, binary_point_o=6, latency=0, overflow=Wrap, quantization=Truncate}
      mask prompts: bit_width_i "Bit Width In"; binary_point_i "Binary Point In"; bit_width_o "Bit Width Out"; binary_point_o "Binary Point Out"; overflow "Overflow Behaviour"; quantization "Quantization Behaviour"
      mask help:
      | Converts from one 2's complement bit-width
      | and/or binary point position to another.
      | Includes underflow/overflow indicator.
      mask init: same as casper_library_correlator/cross_multiplier/cvrt0_0_0_imag
      settings: AttributesFormatString=[9,6]->[9,6]
      mask TypeOptions overflow: Wrap | Saturate | Error
      mask TypeOptions quantization: Truncate | Round  (unbiased: +/- Inf) | Round  (unbiased: even values)
  cvrt3_1_1_real : Subsystem  AncestorBlock=casper_library_misc/convert_of  mask(convert_of){bit_width_i=9, binary_point_i=6, bit_width_o=9, binary_point_o=6, latency=0, overflow=Wrap, quantization=Truncate}
      mask prompts: bit_width_i "Bit Width In"; binary_point_i "Binary Point In"; bit_width_o "Bit Width Out"; binary_point_o "Binary Point Out"; overflow "Overflow Behaviour"; quantization "Quantization Behaviour"
      mask help:
      | Converts from one 2's complement bit-width
      | and/or binary point position to another.
      | Includes underflow/overflow indicator.
      mask init: same as casper_library_correlator/cross_multiplier/cvrt0_0_0_imag
      settings: AttributesFormatString=[9,6]->[9,6]
      mask TypeOptions overflow: Wrap | Saturate | Error
      mask TypeOptions quantization: Truncate | Round  (unbiased: +/- Inf) | Round  (unbiased: even values)
  cvrt3_2_0_imag : Subsystem  AncestorBlock=casper_library_misc/convert_of  mask(convert_of){bit_width_i=9, binary_point_i=6, bit_width_o=9, binary_point_o=6, latency=0, overflow=Wrap, quantization=Truncate}
      mask prompts: bit_width_i "Bit Width In"; binary_point_i "Binary Point In"; bit_width_o "Bit Width Out"; binary_point_o "Binary Point Out"; overflow "Overflow Behaviour"; quantization "Quantization Behaviour"
      mask help:
      | Converts from one 2's complement bit-width
      | and/or binary point position to another.
      | Includes underflow/overflow indicator.
      mask init: same as casper_library_correlator/cross_multiplier/cvrt0_0_0_imag
      settings: AttributesFormatString=[9,6]->[9,6]
      mask TypeOptions overflow: Wrap | Saturate | Error
      mask TypeOptions quantization: Truncate | Round  (unbiased: +/- Inf) | Round  (unbiased: even values)
  cvrt3_2_0_real : Subsystem  AncestorBlock=casper_library_misc/convert_of  mask(convert_of){bit_width_i=9, binary_point_i=6, bit_width_o=9, binary_point_o=6, latency=0, overflow=Wrap, quantization=Truncate}
      mask prompts: bit_width_i "Bit Width In"; binary_point_i "Binary Point In"; bit_width_o "Bit Width Out"; binary_point_o "Binary Point Out"; overflow "Overflow Behaviour"; quantization "Quantization Behaviour"
      mask help:
      | Converts from one 2's complement bit-width
      | and/or binary point position to another.
      | Includes underflow/overflow indicator.
      mask init: same as casper_library_correlator/cross_multiplier/cvrt0_0_0_imag
      settings: AttributesFormatString=[9,6]->[9,6]
      mask TypeOptions overflow: Wrap | Saturate | Error
      mask TypeOptions quantization: Truncate | Round  (unbiased: +/- Inf) | Round  (unbiased: even values)
  cvrt3_2_1_imag : Subsystem  AncestorBlock=casper_library_misc/convert_of  mask(convert_of){bit_width_i=9, binary_point_i=6, bit_width_o=9, binary_point_o=6, latency=0, overflow=Wrap, quantization=Truncate}
      mask prompts: bit_width_i "Bit Width In"; binary_point_i "Binary Point In"; bit_width_o "Bit Width Out"; binary_point_o "Binary Point Out"; overflow "Overflow Behaviour"; quantization "Quantization Behaviour"
      mask help:
      | Converts from one 2's complement bit-width
      | and/or binary point position to another.
      | Includes underflow/overflow indicator.
      mask init: same as casper_library_correlator/cross_multiplier/cvrt0_0_0_imag
      settings: AttributesFormatString=[9,6]->[9,6]
      mask TypeOptions overflow: Wrap | Saturate | Error
      mask TypeOptions quantization: Truncate | Round  (unbiased: +/- Inf) | Round  (unbiased: even values)
  cvrt3_2_1_real : Subsystem  AncestorBlock=casper_library_misc/convert_of  mask(convert_of){bit_width_i=9, binary_point_i=6, bit_width_o=9, binary_point_o=6, latency=0, overflow=Wrap, quantization=Truncate}
      mask prompts: bit_width_i "Bit Width In"; binary_point_i "Binary Point In"; bit_width_o "Bit Width Out"; binary_point_o "Binary Point Out"; overflow "Overflow Behaviour"; quantization "Quantization Behaviour"
      mask help:
      | Converts from one 2's complement bit-width
      | and/or binary point position to another.
      | Includes underflow/overflow indicator.
      mask init: same as casper_library_correlator/cross_multiplier/cvrt0_0_0_imag
      settings: AttributesFormatString=[9,6]->[9,6]
      mask TypeOptions overflow: Wrap | Saturate | Error
      mask TypeOptions quantization: Truncate | Round  (unbiased: +/- Inf) | Round  (unbiased: even values)
  cvrt3_3_0_imag : Subsystem  AncestorBlock=casper_library_misc/convert_of  mask(convert_of){bit_width_i=9, binary_point_i=6, bit_width_o=9, binary_point_o=6, latency=0, overflow=Wrap, quantization=Truncate}
      mask prompts: bit_width_i "Bit Width In"; binary_point_i "Binary Point In"; bit_width_o "Bit Width Out"; binary_point_o "Binary Point Out"; overflow "Overflow Behaviour"; quantization "Quantization Behaviour"
      mask help:
      | Converts from one 2's complement bit-width
      | and/or binary point position to another.
      | Includes underflow/overflow indicator.
      mask init: same as casper_library_correlator/cross_multiplier/cvrt0_0_0_imag
      settings: AttributesFormatString=[9,6]->[9,6]
      mask TypeOptions overflow: Wrap | Saturate | Error
      mask TypeOptions quantization: Truncate | Round  (unbiased: +/- Inf) | Round  (unbiased: even values)
  cvrt3_3_0_real : Subsystem  AncestorBlock=casper_library_misc/convert_of  mask(convert_of){bit_width_i=9, binary_point_i=6, bit_width_o=9, binary_point_o=6, latency=0, overflow=Wrap, quantization=Truncate}
      mask prompts: bit_width_i "Bit Width In"; binary_point_i "Binary Point In"; bit_width_o "Bit Width Out"; binary_point_o "Binary Point Out"; overflow "Overflow Behaviour"; quantization "Quantization Behaviour"
      mask help:
      | Converts from one 2's complement bit-width
      | and/or binary point position to another.
      | Includes underflow/overflow indicator.
      mask init: same as casper_library_correlator/cross_multiplier/cvrt0_0_0_imag
      settings: AttributesFormatString=[9,6]->[9,6]
      mask TypeOptions overflow: Wrap | Saturate | Error
      mask TypeOptions quantization: Truncate | Round  (unbiased: +/- Inf) | Round  (unbiased: even values)
  cvrt3_3_1_imag : Subsystem  AncestorBlock=casper_library_misc/convert_of  mask(convert_of){bit_width_i=9, binary_point_i=6, bit_width_o=9, binary_point_o=6, latency=0, overflow=Wrap, quantization=Truncate}
      mask prompts: bit_width_i "Bit Width In"; binary_point_i "Binary Point In"; bit_width_o "Bit Width Out"; binary_point_o "Binary Point Out"; overflow "Overflow Behaviour"; quantization "Quantization Behaviour"
      mask help:
      | Converts from one 2's complement bit-width
      | and/or binary point position to another.
      | Includes underflow/overflow indicator.
      mask init: same as casper_library_correlator/cross_multiplier/cvrt0_0_0_imag
      settings: AttributesFormatString=[9,6]->[9,6]
      mask TypeOptions overflow: Wrap | Saturate | Error
      mask TypeOptions quantization: Truncate | Round  (unbiased: +/- Inf) | Round  (unbiased: even values)
  cvrt3_3_1_real : Subsystem  AncestorBlock=casper_library_misc/convert_of  mask(convert_of){bit_width_i=9, binary_point_i=6, bit_width_o=9, binary_point_o=6, latency=0, overflow=Wrap, quantization=Truncate}
      mask prompts: bit_width_i "Bit Width In"; binary_point_i "Binary Point In"; bit_width_o "Bit Width Out"; binary_point_o "Binary Point Out"; overflow "Overflow Behaviour"; quantization "Quantization Behaviour"
      mask help:
      | Converts from one 2's complement bit-width
      | and/or binary point position to another.
      | Includes underflow/overflow indicator.
      mask init: same as casper_library_correlator/cross_multiplier/cvrt0_0_0_imag
      settings: AttributesFormatString=[9,6]->[9,6]
      mask TypeOptions overflow: Wrap | Saturate | Error
      mask TypeOptions quantization: Truncate | Round  (unbiased: +/- Inf) | Round  (unbiased: even values)
  cvrt3_4_0_imag : Subsystem  AncestorBlock=casper_library_misc/convert_of  mask(convert_of){bit_width_i=9, binary_point_i=6, bit_width_o=9, binary_point_o=6, latency=0, overflow=Wrap, quantization=Truncate}
      mask prompts: bit_width_i "Bit Width In"; binary_point_i "Binary Point In"; bit_width_o "Bit Width Out"; binary_point_o "Binary Point Out"; overflow "Overflow Behaviour"; quantization "Quantization Behaviour"
      mask help:
      | Converts from one 2's complement bit-width
      | and/or binary point position to another.
      | Includes underflow/overflow indicator.
      mask init: same as casper_library_correlator/cross_multiplier/cvrt0_0_0_imag
      settings: AttributesFormatString=[9,6]->[9,6]
      mask TypeOptions overflow: Wrap | Saturate | Error
      mask TypeOptions quantization: Truncate | Round  (unbiased: +/- Inf) | Round  (unbiased: even values)
  cvrt3_4_0_real : Subsystem  AncestorBlock=casper_library_misc/convert_of  mask(convert_of){bit_width_i=9, binary_point_i=6, bit_width_o=9, binary_point_o=6, latency=0, overflow=Wrap, quantization=Truncate}
      mask prompts: bit_width_i "Bit Width In"; binary_point_i "Binary Point In"; bit_width_o "Bit Width Out"; binary_point_o "Binary Point Out"; overflow "Overflow Behaviour"; quantization "Quantization Behaviour"
      mask help:
      | Converts from one 2's complement bit-width
      | and/or binary point position to another.
      | Includes underflow/overflow indicator.
      mask init: same as casper_library_correlator/cross_multiplier/cvrt0_0_0_imag
      settings: AttributesFormatString=[9,6]->[9,6]
      mask TypeOptions overflow: Wrap | Saturate | Error
      mask TypeOptions quantization: Truncate | Round  (unbiased: +/- Inf) | Round  (unbiased: even values)
  cvrt3_4_1_imag : Subsystem  AncestorBlock=casper_library_misc/convert_of  mask(convert_of){bit_width_i=9, binary_point_i=6, bit_width_o=9, binary_point_o=6, latency=0, overflow=Wrap, quantization=Truncate}
      mask prompts: bit_width_i "Bit Width In"; binary_point_i "Binary Point In"; bit_width_o "Bit Width Out"; binary_point_o "Binary Point Out"; overflow "Overflow Behaviour"; quantization "Quantization Behaviour"
      mask help:
      | Converts from one 2's complement bit-width
      | and/or binary point position to another.
      | Includes underflow/overflow indicator.
      mask init: same as casper_library_correlator/cross_multiplier/cvrt0_0_0_imag
      settings: AttributesFormatString=[9,6]->[9,6]
      mask TypeOptions overflow: Wrap | Saturate | Error
      mask TypeOptions quantization: Truncate | Round  (unbiased: +/- Inf) | Round  (unbiased: even values)
  cvrt3_4_1_real : Subsystem  AncestorBlock=casper_library_misc/convert_of  mask(convert_of){bit_width_i=9, binary_point_i=6, bit_width_o=9, binary_point_o=6, latency=0, overflow=Wrap, quantization=Truncate}
      mask prompts: bit_width_i "Bit Width In"; binary_point_i "Binary Point In"; bit_width_o "Bit Width Out"; binary_point_o "Binary Point Out"; overflow "Overflow Behaviour"; quantization "Quantization Behaviour"
      mask help:
      | Converts from one 2's complement bit-width
      | and/or binary point position to another.
      | Includes underflow/overflow indicator.
      mask init: same as casper_library_correlator/cross_multiplier/cvrt0_0_0_imag
      settings: AttributesFormatString=[9,6]->[9,6]
      mask TypeOptions overflow: Wrap | Saturate | Error
      mask TypeOptions quantization: Truncate | Round  (unbiased: +/- Inf) | Round  (unbiased: even values)
  cvrt3_5_0_imag : Subsystem  AncestorBlock=casper_library_misc/convert_of  mask(convert_of){bit_width_i=9, binary_point_i=6, bit_width_o=9, binary_point_o=6, latency=0, overflow=Wrap, quantization=Truncate}
      mask prompts: bit_width_i "Bit Width In"; binary_point_i "Binary Point In"; bit_width_o "Bit Width Out"; binary_point_o "Binary Point Out"; overflow "Overflow Behaviour"; quantization "Quantization Behaviour"
      mask help:
      | Converts from one 2's complement bit-width
      | and/or binary point position to another.
      | Includes underflow/overflow indicator.
      mask init: same as casper_library_correlator/cross_multiplier/cvrt0_0_0_imag
      settings: AttributesFormatString=[9,6]->[9,6]
      mask TypeOptions overflow: Wrap | Saturate | Error
      mask TypeOptions quantization: Truncate | Round  (unbiased: +/- Inf) | Round  (unbiased: even values)
  cvrt3_5_0_real : Subsystem  AncestorBlock=casper_library_misc/convert_of  mask(convert_of){bit_width_i=9, binary_point_i=6, bit_width_o=9, binary_point_o=6, latency=0, overflow=Wrap, quantization=Truncate}
      mask prompts: bit_width_i "Bit Width In"; binary_point_i "Binary Point In"; bit_width_o "Bit Width Out"; binary_point_o "Binary Point Out"; overflow "Overflow Behaviour"; quantization "Quantization Behaviour"
      mask help:
      | Converts from one 2's complement bit-width
      | and/or binary point position to another.
      | Includes underflow/overflow indicator.
      mask init: same as casper_library_correlator/cross_multiplier/cvrt0_0_0_imag
      settings: AttributesFormatString=[9,6]->[9,6]
      mask TypeOptions overflow: Wrap | Saturate | Error
      mask TypeOptions quantization: Truncate | Round  (unbiased: +/- Inf) | Round  (unbiased: even values)
  cvrt3_5_1_imag : Subsystem  AncestorBlock=casper_library_misc/convert_of  mask(convert_of){bit_width_i=9, binary_point_i=6, bit_width_o=9, binary_point_o=6, latency=0, overflow=Wrap, quantization=Truncate}
      mask prompts: bit_width_i "Bit Width In"; binary_point_i "Binary Point In"; bit_width_o "Bit Width Out"; binary_point_o "Binary Point Out"; overflow "Overflow Behaviour"; quantization "Quantization Behaviour"
      mask help:
      | Converts from one 2's complement bit-width
      | and/or binary point position to another.
      | Includes underflow/overflow indicator.
      mask init: same as casper_library_correlator/cross_multiplier/cvrt0_0_0_imag
      settings: AttributesFormatString=[9,6]->[9,6]
      mask TypeOptions overflow: Wrap | Saturate | Error
      mask TypeOptions quantization: Truncate | Round  (unbiased: +/- Inf) | Round  (unbiased: even values)
  cvrt3_5_1_real : Subsystem  AncestorBlock=casper_library_misc/convert_of  mask(convert_of){bit_width_i=9, binary_point_i=6, bit_width_o=9, binary_point_o=6, latency=0, overflow=Wrap, quantization=Truncate}
      mask prompts: bit_width_i "Bit Width In"; binary_point_i "Binary Point In"; bit_width_o "Bit Width Out"; binary_point_o "Binary Point Out"; overflow "Overflow Behaviour"; quantization "Quantization Behaviour"
      mask help:
      | Converts from one 2's complement bit-width
      | and/or binary point position to another.
      | Includes underflow/overflow indicator.
      mask init: same as casper_library_correlator/cross_multiplier/cvrt0_0_0_imag
      settings: AttributesFormatString=[9,6]->[9,6]
      mask TypeOptions overflow: Wrap | Saturate | Error
      mask TypeOptions quantization: Truncate | Round  (unbiased: +/- Inf) | Round  (unbiased: even values)
  cvrt3_6_0_imag : Subsystem  AncestorBlock=casper_library_misc/convert_of  mask(convert_of){bit_width_i=9, binary_point_i=6, bit_width_o=9, binary_point_o=6, latency=0, overflow=Wrap, quantization=Truncate}
      mask prompts: bit_width_i "Bit Width In"; binary_point_i "Binary Point In"; bit_width_o "Bit Width Out"; binary_point_o "Binary Point Out"; overflow "Overflow Behaviour"; quantization "Quantization Behaviour"
      mask help:
      | Converts from one 2's complement bit-width
      | and/or binary point position to another.
      | Includes underflow/overflow indicator.
      mask init: same as casper_library_correlator/cross_multiplier/cvrt0_0_0_imag
      settings: AttributesFormatString=[9,6]->[9,6]
      mask TypeOptions overflow: Wrap | Saturate | Error
      mask TypeOptions quantization: Truncate | Round  (unbiased: +/- Inf) | Round  (unbiased: even values)
  cvrt3_6_0_real : Subsystem  AncestorBlock=casper_library_misc/convert_of  mask(convert_of){bit_width_i=9, binary_point_i=6, bit_width_o=9, binary_point_o=6, latency=0, overflow=Wrap, quantization=Truncate}
      mask prompts: bit_width_i "Bit Width In"; binary_point_i "Binary Point In"; bit_width_o "Bit Width Out"; binary_point_o "Binary Point Out"; overflow "Overflow Behaviour"; quantization "Quantization Behaviour"
      mask help:
      | Converts from one 2's complement bit-width
      | and/or binary point position to another.
      | Includes underflow/overflow indicator.
      mask init: same as casper_library_correlator/cross_multiplier/cvrt0_0_0_imag
      settings: AttributesFormatString=[9,6]->[9,6]
      mask TypeOptions overflow: Wrap | Saturate | Error
      mask TypeOptions quantization: Truncate | Round  (unbiased: +/- Inf) | Round  (unbiased: even values)
  cvrt3_6_1_imag : Subsystem  AncestorBlock=casper_library_misc/convert_of  mask(convert_of){bit_width_i=9, binary_point_i=6, bit_width_o=9, binary_point_o=6, latency=0, overflow=Wrap, quantization=Truncate}
      mask prompts: bit_width_i "Bit Width In"; binary_point_i "Binary Point In"; bit_width_o "Bit Width Out"; binary_point_o "Binary Point Out"; overflow "Overflow Behaviour"; quantization "Quantization Behaviour"
      mask help:
      | Converts from one 2's complement bit-width
      | and/or binary point position to another.
      | Includes underflow/overflow indicator.
      mask init: same as casper_library_correlator/cross_multiplier/cvrt0_0_0_imag
      settings: AttributesFormatString=[9,6]->[9,6]
      mask TypeOptions overflow: Wrap | Saturate | Error
      mask TypeOptions quantization: Truncate | Round  (unbiased: +/- Inf) | Round  (unbiased: even values)
  cvrt3_6_1_real : Subsystem  AncestorBlock=casper_library_misc/convert_of  mask(convert_of){bit_width_i=9, binary_point_i=6, bit_width_o=9, binary_point_o=6, latency=0, overflow=Wrap, quantization=Truncate}
      mask prompts: bit_width_i "Bit Width In"; binary_point_i "Binary Point In"; bit_width_o "Bit Width Out"; binary_point_o "Binary Point Out"; overflow "Overflow Behaviour"; quantization "Quantization Behaviour"
      mask help:
      | Converts from one 2's complement bit-width
      | and/or binary point position to another.
      | Includes underflow/overflow indicator.
      mask init: same as casper_library_correlator/cross_multiplier/cvrt0_0_0_imag
      settings: AttributesFormatString=[9,6]->[9,6]
      mask TypeOptions overflow: Wrap | Saturate | Error
      mask TypeOptions quantization: Truncate | Round  (unbiased: +/- Inf) | Round  (unbiased: even values)
  delay0_0_0_{0..3} (4 alike) : xbsIndex_r4/Delay  rst=off  infoeditControl=Selection of Reset will increase slice count due to use of real FFs and instead of SRLs  en=off  latency=1  dbl_ovrd=off  reg_retiming=off  block_type=delay
  delay0_0_1_{0..3} (4 alike) : xbsIndex_r4/Delay  rst=off  infoeditControl=Selection of Reset will increase slice count due to use of real FFs and instead of SRLs  en=off  latency=1  dbl_ovrd=off  reg_retiming=off  block_type=delay
  delay1_0_0_{0..3} (4 alike) : xbsIndex_r4/Delay  rst=off  infoeditControl=Selection of Reset will increase slice count due to use of real FFs and instead of SRLs  en=off  latency=1  dbl_ovrd=off  reg_retiming=off  block_type=delay
  delay1_0_1_{0..3} (4 alike) : xbsIndex_r4/Delay  rst=off  infoeditControl=Selection of Reset will increase slice count due to use of real FFs and instead of SRLs  en=off  latency=1  dbl_ovrd=off  reg_retiming=off  block_type=delay
  delay1_1_0_{0..3} (4 alike) : xbsIndex_r4/Delay  rst=off  infoeditControl=Selection of Reset will increase slice count due to use of real FFs and instead of SRLs  en=off  latency=1  dbl_ovrd=off  reg_retiming=off  block_type=delay
  delay1_1_1_{0..3} (4 alike) : xbsIndex_r4/Delay  rst=off  infoeditControl=Selection of Reset will increase slice count due to use of real FFs and instead of SRLs  en=off  latency=1  dbl_ovrd=off  reg_retiming=off  block_type=delay
  delay1_2_0_{0..3} (4 alike) : xbsIndex_r4/Delay  rst=off  infoeditControl=Selection of Reset will increase slice count due to use of real FFs and instead of SRLs  en=off  latency=1  dbl_ovrd=off  reg_retiming=off  block_type=delay
  delay1_2_1_{0..3} (4 alike) : xbsIndex_r4/Delay  rst=off  infoeditControl=Selection of Reset will increase slice count due to use of real FFs and instead of SRLs  en=off  latency=1  dbl_ovrd=off  reg_retiming=off  block_type=delay
  delay2_0_0_{0..3} (4 alike) : xbsIndex_r4/Delay  rst=off  infoeditControl=Selection of Reset will increase slice count due to use of real FFs and instead of SRLs  en=off  latency=1  dbl_ovrd=off  reg_retiming=off  block_type=delay
  delay2_0_1_{0..3} (4 alike) : xbsIndex_r4/Delay  rst=off  infoeditControl=Selection of Reset will increase slice count due to use of real FFs and instead of SRLs  en=off  latency=1  dbl_ovrd=off  reg_retiming=off  block_type=delay
  delay2_1_0_{0..3} (4 alike) : xbsIndex_r4/Delay  rst=off  infoeditControl=Selection of Reset will increase slice count due to use of real FFs and instead of SRLs  en=off  latency=1  dbl_ovrd=off  reg_retiming=off  block_type=delay
  delay2_1_1_{0..3} (4 alike) : xbsIndex_r4/Delay  rst=off  infoeditControl=Selection of Reset will increase slice count due to use of real FFs and instead of SRLs  en=off  latency=1  dbl_ovrd=off  reg_retiming=off  block_type=delay
  delay2_2_0_{0..3} (4 alike) : xbsIndex_r4/Delay  rst=off  infoeditControl=Selection of Reset will increase slice count due to use of real FFs and instead of SRLs  en=off  latency=1  dbl_ovrd=off  reg_retiming=off  block_type=delay
  delay2_2_1_{0..3} (4 alike) : xbsIndex_r4/Delay  rst=off  infoeditControl=Selection of Reset will increase slice count due to use of real FFs and instead of SRLs  en=off  latency=1  dbl_ovrd=off  reg_retiming=off  block_type=delay
  delay2_3_0_{0..3} (4 alike) : xbsIndex_r4/Delay  rst=off  infoeditControl=Selection of Reset will increase slice count due to use of real FFs and instead of SRLs  en=off  latency=1  dbl_ovrd=off  reg_retiming=off  block_type=delay
  delay2_3_1_{0..3} (4 alike) : xbsIndex_r4/Delay  rst=off  infoeditControl=Selection of Reset will increase slice count due to use of real FFs and instead of SRLs  en=off  latency=1  dbl_ovrd=off  reg_retiming=off  block_type=delay
  delay2_4_0_{0..3} (4 alike) : xbsIndex_r4/Delay  rst=off  infoeditControl=Selection of Reset will increase slice count due to use of real FFs and instead of SRLs  en=off  latency=1  dbl_ovrd=off  reg_retiming=off  block_type=delay
  delay2_4_1_{0..3} (4 alike) : xbsIndex_r4/Delay  rst=off  infoeditControl=Selection of Reset will increase slice count due to use of real FFs and instead of SRLs  en=off  latency=1  dbl_ovrd=off  reg_retiming=off  block_type=delay
  delay3_0_0_{0..3} (4 alike) : xbsIndex_r4/Delay  rst=off  infoeditControl=Selection of Reset will increase slice count due to use of real FFs and instead of SRLs  en=off  latency=1  dbl_ovrd=off  reg_retiming=off  block_type=delay
  delay3_0_1_{0..3} (4 alike) : xbsIndex_r4/Delay  rst=off  infoeditControl=Selection of Reset will increase slice count due to use of real FFs and instead of SRLs  en=off  latency=1  dbl_ovrd=off  reg_retiming=off  block_type=delay
  delay3_1_0_{0..3} (4 alike) : xbsIndex_r4/Delay  rst=off  infoeditControl=Selection of Reset will increase slice count due to use of real FFs and instead of SRLs  en=off  latency=1  dbl_ovrd=off  reg_retiming=off  block_type=delay
  delay3_1_1_{0..3} (4 alike) : xbsIndex_r4/Delay  rst=off  infoeditControl=Selection of Reset will increase slice count due to use of real FFs and instead of SRLs  en=off  latency=1  dbl_ovrd=off  reg_retiming=off  block_type=delay
  delay3_2_0_{0..3} (4 alike) : xbsIndex_r4/Delay  rst=off  infoeditControl=Selection of Reset will increase slice count due to use of real FFs and instead of SRLs  en=off  latency=1  dbl_ovrd=off  reg_retiming=off  block_type=delay
  delay3_2_1_{0..3} (4 alike) : xbsIndex_r4/Delay  rst=off  infoeditControl=Selection of Reset will increase slice count due to use of real FFs and instead of SRLs  en=off  latency=1  dbl_ovrd=off  reg_retiming=off  block_type=delay
  delay3_3_0_{0..3} (4 alike) : xbsIndex_r4/Delay  rst=off  infoeditControl=Selection of Reset will increase slice count due to use of real FFs and instead of SRLs  en=off  latency=1  dbl_ovrd=off  reg_retiming=off  block_type=delay
  delay3_3_1_{0..3} (4 alike) : xbsIndex_r4/Delay  rst=off  infoeditControl=Selection of Reset will increase slice count due to use of real FFs and instead of SRLs  en=off  latency=1  dbl_ovrd=off  reg_retiming=off  block_type=delay
  delay3_4_0_{0..3} (4 alike) : xbsIndex_r4/Delay  rst=off  infoeditControl=Selection of Reset will increase slice count due to use of real FFs and instead of SRLs  en=off  latency=1  dbl_ovrd=off  reg_retiming=off  block_type=delay
  delay3_4_1_{0..3} (4 alike) : xbsIndex_r4/Delay  rst=off  infoeditControl=Selection of Reset will increase slice count due to use of real FFs and instead of SRLs  en=off  latency=1  dbl_ovrd=off  reg_retiming=off  block_type=delay
  delay3_5_0_{0..3} (4 alike) : xbsIndex_r4/Delay  rst=off  infoeditControl=Selection of Reset will increase slice count due to use of real FFs and instead of SRLs  en=off  latency=1  dbl_ovrd=off  reg_retiming=off  block_type=delay
  delay3_5_1_{0..3} (4 alike) : xbsIndex_r4/Delay  rst=off  infoeditControl=Selection of Reset will increase slice count due to use of real FFs and instead of SRLs  en=off  latency=1  dbl_ovrd=off  reg_retiming=off  block_type=delay
  delay3_6_0_{0..3} (4 alike) : xbsIndex_r4/Delay  rst=off  infoeditControl=Selection of Reset will increase slice count due to use of real FFs and instead of SRLs  en=off  latency=1  dbl_ovrd=off  reg_retiming=off  block_type=delay
  delay3_6_1_{0..3} (4 alike) : xbsIndex_r4/Delay  rst=off  infoeditControl=Selection of Reset will increase slice count due to use of real FFs and instead of SRLs  en=off  latency=1  dbl_ovrd=off  reg_retiming=off  block_type=delay
  pack0_0 : Subsystem  AncestorBlock=gavrt_library/cram  mask(cram){num_slice=aggregation}
      mask prompts: num_slice "Number of slices"
      mask help: Concatenates inputs together after forcing binary point to zero.
      mask init:
      | cram_init(gcb, ...
      |     'num_slice', num_slice);
  pack1_0 : Subsystem  AncestorBlock=gavrt_library/cram  mask(cram){num_slice=aggregation}
      mask prompts: num_slice "Number of slices"
      mask help: Concatenates inputs together after forcing binary point to zero.
      mask init:
      | cram_init(gcb, ...
      |     'num_slice', num_slice);
  pack1_1 : Subsystem  AncestorBlock=gavrt_library/cram  mask(cram){num_slice=aggregation}
      mask prompts: num_slice "Number of slices"
      mask help: Concatenates inputs together after forcing binary point to zero.
      mask init:
      | cram_init(gcb, ...
      |     'num_slice', num_slice);
  pack1_2 : Subsystem  AncestorBlock=gavrt_library/cram  mask(cram){num_slice=aggregation}
      mask prompts: num_slice "Number of slices"
      mask help: Concatenates inputs together after forcing binary point to zero.
      mask init:
      | cram_init(gcb, ...
      |     'num_slice', num_slice);
  pack2_0 : Subsystem  AncestorBlock=gavrt_library/cram  mask(cram){num_slice=aggregation}
      mask prompts: num_slice "Number of slices"
      mask help: Concatenates inputs together after forcing binary point to zero.
      mask init:
      | cram_init(gcb, ...
      |     'num_slice', num_slice);
  pack2_1 : Subsystem  AncestorBlock=gavrt_library/cram  mask(cram){num_slice=aggregation}
      mask prompts: num_slice "Number of slices"
      mask help: Concatenates inputs together after forcing binary point to zero.
      mask init:
      | cram_init(gcb, ...
      |     'num_slice', num_slice);
  pack2_2 : Subsystem  AncestorBlock=gavrt_library/cram  mask(cram){num_slice=aggregation}
      mask prompts: num_slice "Number of slices"
      mask help: Concatenates inputs together after forcing binary point to zero.
      mask init:
      | cram_init(gcb, ...
      |     'num_slice', num_slice);
  pack2_3 : Subsystem  AncestorBlock=gavrt_library/cram  mask(cram){num_slice=aggregation}
      mask prompts: num_slice "Number of slices"
      mask help: Concatenates inputs together after forcing binary point to zero.
      mask init:
      | cram_init(gcb, ...
      |     'num_slice', num_slice);
  pack2_4 : Subsystem  AncestorBlock=gavrt_library/cram  mask(cram){num_slice=aggregation}
      mask prompts: num_slice "Number of slices"
      mask help: Concatenates inputs together after forcing binary point to zero.
      mask init:
      | cram_init(gcb, ...
      |     'num_slice', num_slice);
  pack3_0 : Subsystem  AncestorBlock=gavrt_library/cram  mask(cram){num_slice=aggregation}
      mask prompts: num_slice "Number of slices"
      mask help: Concatenates inputs together after forcing binary point to zero.
      mask init:
      | cram_init(gcb, ...
      |     'num_slice', num_slice);
  pack3_1 : Subsystem  AncestorBlock=gavrt_library/cram  mask(cram){num_slice=aggregation}
      mask prompts: num_slice "Number of slices"
      mask help: Concatenates inputs together after forcing binary point to zero.
      mask init:
      | cram_init(gcb, ...
      |     'num_slice', num_slice);
  pack3_2 : Subsystem  AncestorBlock=gavrt_library/cram  mask(cram){num_slice=aggregation}
      mask prompts: num_slice "Number of slices"
      mask help: Concatenates inputs together after forcing binary point to zero.
      mask init:
      | cram_init(gcb, ...
      |     'num_slice', num_slice);
  pack3_3 : Subsystem  AncestorBlock=gavrt_library/cram  mask(cram){num_slice=aggregation}
      mask prompts: num_slice "Number of slices"
      mask help: Concatenates inputs together after forcing binary point to zero.
      mask init:
      | cram_init(gcb, ...
      |     'num_slice', num_slice);
  pack3_4 : Subsystem  AncestorBlock=gavrt_library/cram  mask(cram){num_slice=aggregation}
      mask prompts: num_slice "Number of slices"
      mask help: Concatenates inputs together after forcing binary point to zero.
      mask init:
      | cram_init(gcb, ...
      |     'num_slice', num_slice);
  pack3_5 : Subsystem  AncestorBlock=gavrt_library/cram  mask(cram){num_slice=aggregation}
      mask prompts: num_slice "Number of slices"
      mask help: Concatenates inputs together after forcing binary point to zero.
      mask init:
      | cram_init(gcb, ...
      |     'num_slice', num_slice);
  pack3_6 : Subsystem  AncestorBlock=gavrt_library/cram  mask(cram){num_slice=aggregation}
      mask prompts: num_slice "Number of slices"
      mask help: Concatenates inputs together after forcing binary point to zero.
      mask init:
      | cram_init(gcb, ...
      |     'num_slice', num_slice);
  ri_to_c0_0_0 : casper_library_misc/ri_to_c
  ri_to_c0_0_1 : casper_library_misc/ri_to_c
  ri_to_c1_0_0 : casper_library_misc/ri_to_c
  ri_to_c1_0_1 : casper_library_misc/ri_to_c
  ri_to_c1_1_0 : casper_library_misc/ri_to_c
  ri_to_c1_1_1 : casper_library_misc/ri_to_c
  ri_to_c1_2_0 : casper_library_misc/ri_to_c
  ri_to_c1_2_1 : casper_library_misc/ri_to_c
  ri_to_c2_0_0 : casper_library_misc/ri_to_c
  ri_to_c2_0_1 : casper_library_misc/ri_to_c
  ri_to_c2_1_0 : casper_library_misc/ri_to_c
  ri_to_c2_1_1 : casper_library_misc/ri_to_c
  ri_to_c2_2_0 : casper_library_misc/ri_to_c
  ri_to_c2_2_1 : casper_library_misc/ri_to_c
  ri_to_c2_3_0 : casper_library_misc/ri_to_c
  ri_to_c2_3_1 : casper_library_misc/ri_to_c
  ri_to_c2_4_0 : casper_library_misc/ri_to_c
  ri_to_c2_4_1 : casper_library_misc/ri_to_c
  ri_to_c3_0_0 : casper_library_misc/ri_to_c
  ri_to_c3_0_1 : casper_library_misc/ri_to_c
  ri_to_c3_1_0 : casper_library_misc/ri_to_c
  ri_to_c3_1_1 : casper_library_misc/ri_to_c
  ri_to_c3_2_0 : casper_library_misc/ri_to_c
  ri_to_c3_2_1 : casper_library_misc/ri_to_c
  ri_to_c3_3_0 : casper_library_misc/ri_to_c
  ri_to_c3_3_1 : casper_library_misc/ri_to_c
  ri_to_c3_4_0 : casper_library_misc/ri_to_c
  ri_to_c3_4_1 : casper_library_misc/ri_to_c
  ri_to_c3_5_0 : casper_library_misc/ri_to_c
  ri_to_c3_5_1 : casper_library_misc/ri_to_c
  ri_to_c3_6_0 : casper_library_misc/ri_to_c
  ri_to_c3_6_1 : casper_library_misc/ri_to_c
  sync_delay : xbsIndex_r4/Delay  rst=off  infoeditControl=Selection of Reset will increase slice count due to use of real FFs and instead of SRLs  en=off  latency=mult_latency+add_latency+1+conv_latency  dbl_ovrd=off  reg_retiming=off  block_type=delay
  unpack0 : Subsystem  AncestorBlock=gavrt_library/uncram  mask(uncram){num_slice=aggregation, slice_width=bit_width_in*2, bin_pt=0, arith_type=0}
      mask prompts: num_slice "Number of slices"; slice_width "Slice Width"; bin_pt "Output Binary Point"; arith_type "Output Arithmetic Type (0=Unsigned, 1=Signed)"
      mask help: Takes a concatenated input and slices it up into even pieces and reinterprets them as signed fixed point numbers with a given binary point.
      mask init:
      | uncram_init(gcb, ...
      |     'num_slice', num_slice, ...
      |     'slice_width', slice_width, ...
      |     'bin_pt', bin_pt, ...
      |     'arith_type', arith_type);
      settings: AttributesFormatString=UFix_8_0
  unpack1 : Subsystem  AncestorBlock=gavrt_library/uncram  mask(uncram){num_slice=aggregation, slice_width=bit_width_in*2, bin_pt=0, arith_type=0}
      mask prompts: num_slice "Number of slices"; slice_width "Slice Width"; bin_pt "Output Binary Point"; arith_type "Output Arithmetic Type (0=Unsigned, 1=Signed)"
      mask help: Takes a concatenated input and slices it up into even pieces and reinterprets them as signed fixed point numbers with a given binary point.
      mask init:
      | uncram_init(gcb, ...
      |     'num_slice', num_slice, ...
      |     'slice_width', slice_width, ...
      |     'bin_pt', bin_pt, ...
      |     'arith_type', arith_type);
      settings: AttributesFormatString=UFix_8_0
  unpack2 : Subsystem  AncestorBlock=gavrt_library/uncram  mask(uncram){num_slice=aggregation, slice_width=bit_width_in*2, bin_pt=0, arith_type=0}
      mask prompts: num_slice "Number of slices"; slice_width "Slice Width"; bin_pt "Output Binary Point"; arith_type "Output Arithmetic Type (0=Unsigned, 1=Signed)"
      mask help: Takes a concatenated input and slices it up into even pieces and reinterprets them as signed fixed point numbers with a given binary point.
      mask init:
      | uncram_init(gcb, ...
      |     'num_slice', num_slice, ...
      |     'slice_width', slice_width, ...
      |     'bin_pt', bin_pt, ...
      |     'arith_type', arith_type);
      settings: AttributesFormatString=UFix_8_0
  unpack3 : Subsystem  AncestorBlock=gavrt_library/uncram  mask(uncram){num_slice=aggregation, slice_width=bit_width_in*2, bin_pt=0, arith_type=0}
      mask prompts: num_slice "Number of slices"; slice_width "Slice Width"; bin_pt "Output Binary Point"; arith_type "Output Arithmetic Type (0=Unsigned, 1=Signed)"
      mask help: Takes a concatenated input and slices it up into even pieces and reinterprets them as signed fixed point numbers with a given binary point.
      mask init:
      | uncram_init(gcb, ...
      |     'num_slice', num_slice, ...
      |     'slice_width', slice_width, ...
      |     'bin_pt', bin_pt, ...
      |     'arith_type', arith_type);
      settings: AttributesFormatString=UFix_8_0
  sync_out : Outport
  din0_x_din0* : Outport  Port=2
  din0_x_din1* : Outport  Port=3
  din1_x_din1* : Outport  Port=4
  din1_x_din0* : Outport  Port=5
  din0_x_din2* : Outport  Port=6
  din1_x_din2* : Outport  Port=7
  din2_x_din2* : Outport  Port=8
  din2_x_din1* : Outport  Port=9
  din2_x_din0* : Outport  Port=10
  din0_x_din3* : Outport  Port=11
  din1_x_din3* : Outport  Port=12
  din2_x_din3* : Outport  Port=13
  din3_x_din3* : Outport  Port=14
  din3_x_din2* : Outport  Port=15
  din3_x_din1* : Outport  Port=16
  din3_x_din0* : Outport  Port=17
  wires:
  sync_in/1 -> sync_delay/1
  sync_delay/1 -> sync_out/1
  din0/1 -> unpack0/1(In)
  unpack0/1(Out1) -> c_to_ri0_0/1
  unpack0/2(Out2) -> c_to_ri0_1/1
  c_to_ri0_0/1 -> delay0_0_0_0/1, delay0_0_0_2/1, delay1_0_0_0/1, delay1_2_0_2/1, delay2_0_0_0/1, delay2_4_0_2/1, delay3_0_0_0/1, delay3_6_0_2/1
  delay0_0_0_0/1 -> cmult0_0_0/1
  c_to_ri0_0/2 -> delay0_0_0_1/1, delay0_0_0_3/1, delay1_0_0_1/1, delay1_2_0_3/1, delay2_0_0_1/1, delay2_4_0_3/1, delay3_0_0_1/1, delay3_6_0_3/1
  delay0_0_0_1/1 -> cmult0_0_0/2
  delay0_0_0_2/1 -> cmult0_0_0/3
  delay0_0_0_3/1 -> cmult0_0_0/4
  cmult0_0_0/1 -> cvrt0_0_0_real/1(din)
  cmult0_0_0/2 -> cvrt0_0_0_imag/1(din)
  cvrt0_0_0_real/1(dout) -> ri_to_c0_0_0/1
  cvrt0_0_0_imag/1(dout) -> ri_to_c0_0_0/2
  ri_to_c0_0_0/1 -> pack0_0/1(In1)
  c_to_ri0_1/1 -> delay0_0_1_0/1, delay0_0_1_2/1, delay1_0_1_0/1, delay1_2_1_2/1, delay2_0_1_0/1, delay2_4_1_2/1, delay3_0_1_0/1, delay3_6_1_2/1
  delay0_0_1_0/1 -> cmult0_0_1/1
  c_to_ri0_1/2 -> delay0_0_1_1/1, delay0_0_1_3/1, delay1_0_1_1/1, delay1_2_1_3/1, delay2_0_1_1/1, delay2_4_1_3/1, delay3_0_1_1/1, delay3_6_1_3/1
  delay0_0_1_1/1 -> cmult0_0_1/2
  delay0_0_1_2/1 -> cmult0_0_1/3
  delay0_0_1_3/1 -> cmult0_0_1/4
  cmult0_0_1/1 -> cvrt0_0_1_real/1(din)
  cmult0_0_1/2 -> cvrt0_0_1_imag/1(din)
  cvrt0_0_1_real/1(dout) -> ri_to_c0_0_1/1
  cvrt0_0_1_imag/1(dout) -> ri_to_c0_0_1/2
  ri_to_c0_0_1/1 -> pack0_0/2(In2)
  pack0_0/1(Out) -> din0_x_din0*/1
  din1/1 -> unpack1/1(In)
  unpack1/1(Out1) -> c_to_ri1_0/1
  unpack1/2(Out2) -> c_to_ri1_1/1
  delay1_0_0_0/1 -> cmult1_0_0/1
  delay1_0_0_1/1 -> cmult1_0_0/2
  c_to_ri1_0/1 -> delay1_0_0_2/1, delay1_1_0_0/1, delay1_1_0_2/1, delay1_2_0_0/1, delay2_1_0_0/1, delay2_3_0_2/1, delay3_1_0_0/1, delay3_5_0_2/1
  delay1_0_0_2/1 -> cmult1_0_0/3
  c_to_ri1_0/2 -> delay1_0_0_3/1, delay1_1_0_1/1, delay1_1_0_3/1, delay1_2_0_1/1, delay2_1_0_1/1, delay2_3_0_3/1, delay3_1_0_1/1, delay3_5_0_3/1
  delay1_0_0_3/1 -> cmult1_0_0/4
  cmult1_0_0/1 -> cvrt1_0_0_real/1(din)
  cmult1_0_0/2 -> cvrt1_0_0_imag/1(din)
  cvrt1_0_0_real/1(dout) -> ri_to_c1_0_0/1
  cvrt1_0_0_imag/1(dout) -> ri_to_c1_0_0/2
  ri_to_c1_0_0/1 -> pack1_0/1(In1)
  delay1_0_1_0/1 -> cmult1_0_1/1
  delay1_0_1_1/1 -> cmult1_0_1/2
  c_to_ri1_1/1 -> delay1_0_1_2/1, delay1_1_1_0/1, delay1_1_1_2/1, delay1_2_1_0/1, delay2_1_1_0/1, delay2_3_1_2/1, delay3_1_1_0/1, delay3_5_1_2/1
  delay1_0_1_2/1 -> cmult1_0_1/3
  c_to_ri1_1/2 -> delay1_0_1_3/1, delay1_1_1_1/1, delay1_1_1_3/1, delay1_2_1_1/1, delay2_1_1_1/1, delay2_3_1_3/1, delay3_1_1_1/1, delay3_5_1_3/1
  delay1_0_1_3/1 -> cmult1_0_1/4
  cmult1_0_1/1 -> cvrt1_0_1_real/1(din)
  cmult1_0_1/2 -> cvrt1_0_1_imag/1(din)
  cvrt1_0_1_real/1(dout) -> ri_to_c1_0_1/1
  cvrt1_0_1_imag/1(dout) -> ri_to_c1_0_1/2
  ri_to_c1_0_1/1 -> pack1_0/2(In2)
  pack1_0/1(Out) -> din0_x_din1*/1
  delay1_1_0_0/1 -> cmult1_1_0/1
  delay1_1_0_1/1 -> cmult1_1_0/2
  delay1_1_0_2/1 -> cmult1_1_0/3
  delay1_1_0_3/1 -> cmult1_1_0/4
  cmult1_1_0/1 -> cvrt1_1_0_real/1(din)
  cmult1_1_0/2 -> cvrt1_1_0_imag/1(din)
  cvrt1_1_0_real/1(dout) -> ri_to_c1_1_0/1
  cvrt1_1_0_imag/1(dout) -> ri_to_c1_1_0/2
  ri_to_c1_1_0/1 -> pack1_1/1(In1)
  delay1_1_1_0/1 -> cmult1_1_1/1
  delay1_1_1_1/1 -> cmult1_1_1/2
  delay1_1_1_2/1 -> cmult1_1_1/3
  delay1_1_1_3/1 -> cmult1_1_1/4
  cmult1_1_1/1 -> cvrt1_1_1_real/1(din)
  cmult1_1_1/2 -> cvrt1_1_1_imag/1(din)
  cvrt1_1_1_real/1(dout) -> ri_to_c1_1_1/1
  cvrt1_1_1_imag/1(dout) -> ri_to_c1_1_1/2
  ri_to_c1_1_1/1 -> pack1_1/2(In2)
  pack1_1/1(Out) -> din1_x_din1*/1
  delay1_2_0_0/1 -> cmult1_2_0/1
  delay1_2_0_1/1 -> cmult1_2_0/2
  delay1_2_0_2/1 -> cmult1_2_0/3
  delay1_2_0_3/1 -> cmult1_2_0/4
  cmult1_2_0/1 -> cvrt1_2_0_real/1(din)
  cmult1_2_0/2 -> cvrt1_2_0_imag/1(din)
  cvrt1_2_0_real/1(dout) -> ri_to_c1_2_0/1
  cvrt1_2_0_imag/1(dout) -> ri_to_c1_2_0/2
  ri_to_c1_2_0/1 -> pack1_2/1(In1)
  delay1_2_1_0/1 -> cmult1_2_1/1
  delay1_2_1_1/1 -> cmult1_2_1/2
  delay1_2_1_2/1 -> cmult1_2_1/3
  delay1_2_1_3/1 -> cmult1_2_1/4
  cmult1_2_1/1 -> cvrt1_2_1_real/1(din)
  cmult1_2_1/2 -> cvrt1_2_1_imag/1(din)
  cvrt1_2_1_real/1(dout) -> ri_to_c1_2_1/1
  cvrt1_2_1_imag/1(dout) -> ri_to_c1_2_1/2
  ri_to_c1_2_1/1 -> pack1_2/2(In2)
  pack1_2/1(Out) -> din1_x_din0*/1
  din2/1 -> unpack2/1(In)
  unpack2/1(Out1) -> c_to_ri2_0/1
  unpack2/2(Out2) -> c_to_ri2_1/1
  delay2_0_0_0/1 -> cmult2_0_0/1
  delay2_0_0_1/1 -> cmult2_0_0/2
  c_to_ri2_0/1 -> delay2_0_0_2/1, delay2_1_0_2/1, delay2_2_0_0/1, delay2_2_0_2/1, delay2_3_0_0/1, delay2_4_0_0/1, delay3_2_0_0/1, delay3_4_0_2/1
  delay2_0_0_2/1 -> cmult2_0_0/3
  c_to_ri2_0/2 -> delay2_0_0_3/1, delay2_1_0_3/1, delay2_2_0_1/1, delay2_2_0_3/1, delay2_3_0_1/1, delay2_4_0_1/1, delay3_2_0_1/1, delay3_4_0_3/1
  delay2_0_0_3/1 -> cmult2_0_0/4
  cmult2_0_0/1 -> cvrt2_0_0_real/1(din)
  cmult2_0_0/2 -> cvrt2_0_0_imag/1(din)
  cvrt2_0_0_real/1(dout) -> ri_to_c2_0_0/1
  cvrt2_0_0_imag/1(dout) -> ri_to_c2_0_0/2
  ri_to_c2_0_0/1 -> pack2_0/1(In1)
  delay2_0_1_0/1 -> cmult2_0_1/1
  delay2_0_1_1/1 -> cmult2_0_1/2
  c_to_ri2_1/1 -> delay2_0_1_2/1, delay2_1_1_2/1, delay2_2_1_0/1, delay2_2_1_2/1, delay2_3_1_0/1, delay2_4_1_0/1, delay3_2_1_0/1, delay3_4_1_2/1
  delay2_0_1_2/1 -> cmult2_0_1/3
  c_to_ri2_1/2 -> delay2_0_1_3/1, delay2_1_1_3/1, delay2_2_1_1/1, delay2_2_1_3/1, delay2_3_1_1/1, delay2_4_1_1/1, delay3_2_1_1/1, delay3_4_1_3/1
  delay2_0_1_3/1 -> cmult2_0_1/4
  cmult2_0_1/1 -> cvrt2_0_1_real/1(din)
  cmult2_0_1/2 -> cvrt2_0_1_imag/1(din)
  cvrt2_0_1_real/1(dout) -> ri_to_c2_0_1/1
  cvrt2_0_1_imag/1(dout) -> ri_to_c2_0_1/2
  ri_to_c2_0_1/1 -> pack2_0/2(In2)
  pack2_0/1(Out) -> din0_x_din2*/1
  delay2_1_0_0/1 -> cmult2_1_0/1
  delay2_1_0_1/1 -> cmult2_1_0/2
  delay2_1_0_2/1 -> cmult2_1_0/3
  delay2_1_0_3/1 -> cmult2_1_0/4
  cmult2_1_0/1 -> cvrt2_1_0_real/1(din)
  cmult2_1_0/2 -> cvrt2_1_0_imag/1(din)
  cvrt2_1_0_real/1(dout) -> ri_to_c2_1_0/1
  cvrt2_1_0_imag/1(dout) -> ri_to_c2_1_0/2
  ri_to_c2_1_0/1 -> pack2_1/1(In1)
  delay2_1_1_0/1 -> cmult2_1_1/1
  delay2_1_1_1/1 -> cmult2_1_1/2
  delay2_1_1_2/1 -> cmult2_1_1/3
  delay2_1_1_3/1 -> cmult2_1_1/4
  cmult2_1_1/1 -> cvrt2_1_1_real/1(din)
  cmult2_1_1/2 -> cvrt2_1_1_imag/1(din)
  cvrt2_1_1_real/1(dout) -> ri_to_c2_1_1/1
  cvrt2_1_1_imag/1(dout) -> ri_to_c2_1_1/2
  ri_to_c2_1_1/1 -> pack2_1/2(In2)
  pack2_1/1(Out) -> din1_x_din2*/1
  delay2_2_0_0/1 -> cmult2_2_0/1
  delay2_2_0_1/1 -> cmult2_2_0/2
  delay2_2_0_2/1 -> cmult2_2_0/3
  delay2_2_0_3/1 -> cmult2_2_0/4
  cmult2_2_0/1 -> cvrt2_2_0_real/1(din)
  cmult2_2_0/2 -> cvrt2_2_0_imag/1(din)
  cvrt2_2_0_real/1(dout) -> ri_to_c2_2_0/1
  cvrt2_2_0_imag/1(dout) -> ri_to_c2_2_0/2
  ri_to_c2_2_0/1 -> pack2_2/1(In1)
  delay2_2_1_0/1 -> cmult2_2_1/1
  delay2_2_1_1/1 -> cmult2_2_1/2
  delay2_2_1_2/1 -> cmult2_2_1/3
  delay2_2_1_3/1 -> cmult2_2_1/4
  cmult2_2_1/1 -> cvrt2_2_1_real/1(din)
  cmult2_2_1/2 -> cvrt2_2_1_imag/1(din)
  cvrt2_2_1_real/1(dout) -> ri_to_c2_2_1/1
  cvrt2_2_1_imag/1(dout) -> ri_to_c2_2_1/2
  ri_to_c2_2_1/1 -> pack2_2/2(In2)
  pack2_2/1(Out) -> din2_x_din2*/1
  delay2_3_0_0/1 -> cmult2_3_0/1
  delay2_3_0_1/1 -> cmult2_3_0/2
  delay2_3_0_2/1 -> cmult2_3_0/3
  delay2_3_0_3/1 -> cmult2_3_0/4
  cmult2_3_0/1 -> cvrt2_3_0_real/1(din)
  cmult2_3_0/2 -> cvrt2_3_0_imag/1(din)
  cvrt2_3_0_real/1(dout) -> ri_to_c2_3_0/1
  cvrt2_3_0_imag/1(dout) -> ri_to_c2_3_0/2
  ri_to_c2_3_0/1 -> pack2_3/1(In1)
  delay2_3_1_0/1 -> cmult2_3_1/1
  delay2_3_1_1/1 -> cmult2_3_1/2
  delay2_3_1_2/1 -> cmult2_3_1/3
  delay2_3_1_3/1 -> cmult2_3_1/4
  cmult2_3_1/1 -> cvrt2_3_1_real/1(din)
  cmult2_3_1/2 -> cvrt2_3_1_imag/1(din)
  cvrt2_3_1_real/1(dout) -> ri_to_c2_3_1/1
  cvrt2_3_1_imag/1(dout) -> ri_to_c2_3_1/2
  ri_to_c2_3_1/1 -> pack2_3/2(In2)
  pack2_3/1(Out) -> din2_x_din1*/1
  delay2_4_0_0/1 -> cmult2_4_0/1
  delay2_4_0_1/1 -> cmult2_4_0/2
  delay2_4_0_2/1 -> cmult2_4_0/3
  delay2_4_0_3/1 -> cmult2_4_0/4
  cmult2_4_0/1 -> cvrt2_4_0_real/1(din)
  cmult2_4_0/2 -> cvrt2_4_0_imag/1(din)
  cvrt2_4_0_real/1(dout) -> ri_to_c2_4_0/1
  cvrt2_4_0_imag/1(dout) -> ri_to_c2_4_0/2
  ri_to_c2_4_0/1 -> pack2_4/1(In1)
  delay2_4_1_0/1 -> cmult2_4_1/1
  delay2_4_1_1/1 -> cmult2_4_1/2
  delay2_4_1_2/1 -> cmult2_4_1/3
  delay2_4_1_3/1 -> cmult2_4_1/4
  cmult2_4_1/1 -> cvrt2_4_1_real/1(din)
  cmult2_4_1/2 -> cvrt2_4_1_imag/1(din)
  cvrt2_4_1_real/1(dout) -> ri_to_c2_4_1/1
  cvrt2_4_1_imag/1(dout) -> ri_to_c2_4_1/2
  ri_to_c2_4_1/1 -> pack2_4/2(In2)
  pack2_4/1(Out) -> din2_x_din0*/1
  din3/1 -> unpack3/1(In)
  unpack3/1(Out1) -> c_to_ri3_0/1
  unpack3/2(Out2) -> c_to_ri3_1/1
  delay3_0_0_0/1 -> cmult3_0_0/1
  delay3_0_0_1/1 -> cmult3_0_0/2
  c_to_ri3_0/1 -> delay3_0_0_2/1, delay3_1_0_2/1, delay3_2_0_2/1, delay3_3_0_0/1, delay3_3_0_2/1, delay3_4_0_0/1, delay3_5_0_0/1, delay3_6_0_0/1
  delay3_0_0_2/1 -> cmult3_0_0/3
  c_to_ri3_0/2 -> delay3_0_0_3/1, delay3_1_0_3/1, delay3_2_0_3/1, delay3_3_0_1/1, delay3_3_0_3/1, delay3_4_0_1/1, delay3_5_0_1/1, delay3_6_0_1/1
  delay3_0_0_3/1 -> cmult3_0_0/4
  cmult3_0_0/1 -> cvrt3_0_0_real/1(din)
  cmult3_0_0/2 -> cvrt3_0_0_imag/1(din)
  cvrt3_0_0_real/1(dout) -> ri_to_c3_0_0/1
  cvrt3_0_0_imag/1(dout) -> ri_to_c3_0_0/2
  ri_to_c3_0_0/1 -> pack3_0/1(In1)
  delay3_0_1_0/1 -> cmult3_0_1/1
  delay3_0_1_1/1 -> cmult3_0_1/2
  c_to_ri3_1/1 -> delay3_0_1_2/1, delay3_1_1_2/1, delay3_2_1_2/1, delay3_3_1_0/1, delay3_3_1_2/1, delay3_4_1_0/1, delay3_5_1_0/1, delay3_6_1_0/1
  delay3_0_1_2/1 -> cmult3_0_1/3
  c_to_ri3_1/2 -> delay3_0_1_3/1, delay3_1_1_3/1, delay3_2_1_3/1, delay3_3_1_1/1, delay3_3_1_3/1, delay3_4_1_1/1, delay3_5_1_1/1, delay3_6_1_1/1
  delay3_0_1_3/1 -> cmult3_0_1/4
  cmult3_0_1/1 -> cvrt3_0_1_real/1(din)
  cmult3_0_1/2 -> cvrt3_0_1_imag/1(din)
  cvrt3_0_1_real/1(dout) -> ri_to_c3_0_1/1
  cvrt3_0_1_imag/1(dout) -> ri_to_c3_0_1/2
  ri_to_c3_0_1/1 -> pack3_0/2(In2)
  pack3_0/1(Out) -> din0_x_din3*/1
  delay3_1_0_0/1 -> cmult3_1_0/1
  delay3_1_0_1/1 -> cmult3_1_0/2
  delay3_1_0_2/1 -> cmult3_1_0/3
  delay3_1_0_3/1 -> cmult3_1_0/4
  cmult3_1_0/1 -> cvrt3_1_0_real/1(din)
  cmult3_1_0/2 -> cvrt3_1_0_imag/1(din)
  cvrt3_1_0_real/1(dout) -> ri_to_c3_1_0/1
  cvrt3_1_0_imag/1(dout) -> ri_to_c3_1_0/2
  ri_to_c3_1_0/1 -> pack3_1/1(In1)
  delay3_1_1_0/1 -> cmult3_1_1/1
  delay3_1_1_1/1 -> cmult3_1_1/2
  delay3_1_1_2/1 -> cmult3_1_1/3
  delay3_1_1_3/1 -> cmult3_1_1/4
  cmult3_1_1/1 -> cvrt3_1_1_real/1(din)
  cmult3_1_1/2 -> cvrt3_1_1_imag/1(din)
  cvrt3_1_1_real/1(dout) -> ri_to_c3_1_1/1
  cvrt3_1_1_imag/1(dout) -> ri_to_c3_1_1/2
  ri_to_c3_1_1/1 -> pack3_1/2(In2)
  pack3_1/1(Out) -> din1_x_din3*/1
  delay3_2_0_0/1 -> cmult3_2_0/1
  delay3_2_0_1/1 -> cmult3_2_0/2
  delay3_2_0_2/1 -> cmult3_2_0/3
  delay3_2_0_3/1 -> cmult3_2_0/4
  cmult3_2_0/1 -> cvrt3_2_0_real/1(din)
  cmult3_2_0/2 -> cvrt3_2_0_imag/1(din)
  cvrt3_2_0_real/1(dout) -> ri_to_c3_2_0/1
  cvrt3_2_0_imag/1(dout) -> ri_to_c3_2_0/2
  ri_to_c3_2_0/1 -> pack3_2/1(In1)
  delay3_2_1_0/1 -> cmult3_2_1/1
  delay3_2_1_1/1 -> cmult3_2_1/2
  delay3_2_1_2/1 -> cmult3_2_1/3
  delay3_2_1_3/1 -> cmult3_2_1/4
  cmult3_2_1/1 -> cvrt3_2_1_real/1(din)
  cmult3_2_1/2 -> cvrt3_2_1_imag/1(din)
  cvrt3_2_1_real/1(dout) -> ri_to_c3_2_1/1
  cvrt3_2_1_imag/1(dout) -> ri_to_c3_2_1/2
  ri_to_c3_2_1/1 -> pack3_2/2(In2)
  pack3_2/1(Out) -> din2_x_din3*/1
  delay3_3_0_0/1 -> cmult3_3_0/1
  delay3_3_0_1/1 -> cmult3_3_0/2
  delay3_3_0_2/1 -> cmult3_3_0/3
  delay3_3_0_3/1 -> cmult3_3_0/4
  cmult3_3_0/1 -> cvrt3_3_0_real/1(din)
  cmult3_3_0/2 -> cvrt3_3_0_imag/1(din)
  cvrt3_3_0_real/1(dout) -> ri_to_c3_3_0/1
  cvrt3_3_0_imag/1(dout) -> ri_to_c3_3_0/2
  ri_to_c3_3_0/1 -> pack3_3/1(In1)
  delay3_3_1_0/1 -> cmult3_3_1/1
  delay3_3_1_1/1 -> cmult3_3_1/2
  delay3_3_1_2/1 -> cmult3_3_1/3
  delay3_3_1_3/1 -> cmult3_3_1/4
  cmult3_3_1/1 -> cvrt3_3_1_real/1(din)
  cmult3_3_1/2 -> cvrt3_3_1_imag/1(din)
  cvrt3_3_1_real/1(dout) -> ri_to_c3_3_1/1
  cvrt3_3_1_imag/1(dout) -> ri_to_c3_3_1/2
  ri_to_c3_3_1/1 -> pack3_3/2(In2)
  pack3_3/1(Out) -> din3_x_din3*/1
  delay3_4_0_0/1 -> cmult3_4_0/1
  delay3_4_0_1/1 -> cmult3_4_0/2
  delay3_4_0_2/1 -> cmult3_4_0/3
  delay3_4_0_3/1 -> cmult3_4_0/4
  cmult3_4_0/1 -> cvrt3_4_0_real/1(din)
  cmult3_4_0/2 -> cvrt3_4_0_imag/1(din)
  cvrt3_4_0_real/1(dout) -> ri_to_c3_4_0/1
  cvrt3_4_0_imag/1(dout) -> ri_to_c3_4_0/2
  ri_to_c3_4_0/1 -> pack3_4/1(In1)
  delay3_4_1_0/1 -> cmult3_4_1/1
  delay3_4_1_1/1 -> cmult3_4_1/2
  delay3_4_1_2/1 -> cmult3_4_1/3
  delay3_4_1_3/1 -> cmult3_4_1/4
  cmult3_4_1/1 -> cvrt3_4_1_real/1(din)
  cmult3_4_1/2 -> cvrt3_4_1_imag/1(din)
  cvrt3_4_1_real/1(dout) -> ri_to_c3_4_1/1
  cvrt3_4_1_imag/1(dout) -> ri_to_c3_4_1/2
  ri_to_c3_4_1/1 -> pack3_4/2(In2)
  pack3_4/1(Out) -> din3_x_din2*/1
  delay3_5_0_0/1 -> cmult3_5_0/1
  delay3_5_0_1/1 -> cmult3_5_0/2
  delay3_5_0_2/1 -> cmult3_5_0/3
  delay3_5_0_3/1 -> cmult3_5_0/4
  cmult3_5_0/1 -> cvrt3_5_0_real/1(din)
  cmult3_5_0/2 -> cvrt3_5_0_imag/1(din)
  cvrt3_5_0_real/1(dout) -> ri_to_c3_5_0/1
  cvrt3_5_0_imag/1(dout) -> ri_to_c3_5_0/2
  ri_to_c3_5_0/1 -> pack3_5/1(In1)
  delay3_5_1_0/1 -> cmult3_5_1/1
  delay3_5_1_1/1 -> cmult3_5_1/2
  delay3_5_1_2/1 -> cmult3_5_1/3
  delay3_5_1_3/1 -> cmult3_5_1/4
  cmult3_5_1/1 -> cvrt3_5_1_real/1(din)
  cmult3_5_1/2 -> cvrt3_5_1_imag/1(din)
  cvrt3_5_1_real/1(dout) -> ri_to_c3_5_1/1
  cvrt3_5_1_imag/1(dout) -> ri_to_c3_5_1/2
  ri_to_c3_5_1/1 -> pack3_5/2(In2)
  pack3_5/1(Out) -> din3_x_din1*/1
  delay3_6_0_0/1 -> cmult3_6_0/1
  delay3_6_0_1/1 -> cmult3_6_0/2
  delay3_6_0_2/1 -> cmult3_6_0/3
  delay3_6_0_3/1 -> cmult3_6_0/4
  cmult3_6_0/1 -> cvrt3_6_0_real/1(din)
  cmult3_6_0/2 -> cvrt3_6_0_imag/1(din)
  cvrt3_6_0_real/1(dout) -> ri_to_c3_6_0/1
  cvrt3_6_0_imag/1(dout) -> ri_to_c3_6_0/2
  ri_to_c3_6_0/1 -> pack3_6/1(In1)
  delay3_6_1_0/1 -> cmult3_6_1/1
  delay3_6_1_1/1 -> cmult3_6_1/2
  delay3_6_1_2/1 -> cmult3_6_1/3
  delay3_6_1_3/1 -> cmult3_6_1/4
  cmult3_6_1/1 -> cvrt3_6_1_real/1(din)
  cmult3_6_1/2 -> cvrt3_6_1_imag/1(din)
  cvrt3_6_1_real/1(dout) -> ri_to_c3_6_1/1
  cvrt3_6_1_imag/1(dout) -> ri_to_c3_6_1/2
  ri_to_c3_6_1/1 -> pack3_6/2(In2)
  pack3_6/1(Out) -> din3_x_din0*/1
